simulink model "pwtsimplificado"  (R2025a)
settings: Solver=ode3  StartTime=0.0  StopTime=34  FixedStep=Amostragem/10  RelTol=1e-3
InitFcn:
  | % Suprime os warnings de limite do MFeval. Eles disparam A CADA PASSO quando o pneu
  | % opera fora da faixa do .tir (frenagem forte, baixa velocidade, Fz baixo) e chegam a
  | % custar 10x o tempo de simulacao. Os valores ja sao saturados internamente pelo solver.
  | warning('off','Solver:Limits:Exceeded');
  | warning('off','Solver:CoeffChecks:Ex');
model workspace (MATLAB code in the model file):
  | %% --- Acumulador (lado DC) ----------------------------------------------
  | Bi = 250 ;             % Corrente DC maxima do acumulador (A) - limite de POTENCIA no lado DC.
  |                        %   NAO usar como limite de corrente de fase (ver I_max).
  |                        %   Com 28 kW de pico e EFF ~83%: 234 A @144V -> so 6% de folga.
  | Bv = 168 ;             % Tensao do acumulador (V) - carga cheia (nominal ~144 V)
  | %% --- Motor (identificado a partir das tabelas da folha) ----------------
  | Pnom  = 11000 ;        % Potencia nominal do motor (W)
  | T_max = 94 ;           % Torque maximo/pico 2-min (N*m) - usar na saturacao de Torque_ref
  | Poles = 2 ;            % Numero de PARES de polos (motor de 4 polos -> Poles = 2)
  | Rs  = 0.0165 ;         % Resistencia do estator por fase (Ohm) - folha obs.9: 0.033 de linha /2
  |                        %   (a identificacao usou 0.0144 fixo; diferenca so mexe ~7% no Ki)
  | Rr  = 0.01858 ;        % Resistencia do rotor referida ao estator (Ohm) - IDENTIFICADO
  |                        %   NUNCA usar 0.0248/0.0139: 0.0248 veio do Tau_r=35.5ms
  |                        %   INTERMEDIARIO ERRADO (assumia Kt/Imag antigos); reverter se aparecer.
  | Lls = 7.4763e-5 ;      % Indutancia de dispersao do estator (H) - IDENTIFICADO (Lls=Llr imposto)
  | Llr = 7.4763e-5 ;      % Indutancia de dispersao do rotor (H)   - IDENTIFICADO
  | Lm  = 1.0357e-3 ;      % Indutancia de magnetizacao (H) - IDENTIFICADO (valor LINEAR, fluxo parcial)
  | Ls  = Lls + Lm ;       % Indutancia total do estator (H)  = 1.1105e-3
  | Lr  = Lm + Llr ;       % Indutancia total do rotor (H)    = 1.1105e-3
  | Im  = 0.0071 ;         % Inercia do rotor (kg*m^2). A folha escreve "kgfm2" mas o valor e SI:
  |                        %   carcaca 100 limita o rotor a r<~7cm -> J~0.007-0.01 kg*m^2;
  |                        %   0.0697 (x9.81) exigiria r~12cm, impossivel. [dica: Im=100 trava o rotor]
  | motor_eff = 0.874 ;    % Eficiencia nominal do motor (-) (folha: 87.4% nominal, ~83% no pico)
  | mc_eff    = 0.95 ;     % Eficiencia do inversor (-)
  | %% --- Constantes derivadas do motor -------------------------------------
  | sigma = 1 - (Lm^2)/(Ls*Lr) ;      % Coef. de dispersao total (-)             ~0.1301
  | Tau_r = Lr/Rr ;                   % Constante de tempo do rotor (s)          ~59.8 ms
  |                                   %   Gain "1/Tau_r" embutido no modelo -> 16.73
  | Kt    = (3/2)*Poles*(Lm^2/Lr) ;   % Constante de torque p/ correntes de PICO ~2.898e-3 N*m/A^2
  | Req   = Rs + Rr*((Lm/Lr)^2) ;     % Resistencia equivalente da malha de corrente (Ohm) ~0.0327
  | %% --- Correntes de referencia (PICO de fase) ----------------------------
  | Imag  = 105 ;          % Corrente de magnetizacao (A PICO) - IDENTIFICADA (74 A RMS).
  |                        %   NAO e a "corrente a vazio" da folha (114 RMS = fluxo pleno SATURADO,
  |                        %   fora da regiao linear). Constant "Imag" embutida no modelo -> 105.
  | Idref = Imag ;         % Referencia inicial de corrente do eixo d (A pico)
  | I_max_motor = 242*sqrt(2) ; % Pico 2-min do MOTOR (242 A RMS -> 342.2 pico) - folha
  | I_max_inv   = 257*sqrt(2) ; % Limite AC 1-min do SEVCON Gen5 (257 A RMS -> 363.5 pico)
  | I_max = min(I_max_motor, I_max_inv) ; % limite operativo = o mais restritivo (342.2 pico)
  | % Iq_sat e calculado DINAMICAMENTE no modelo: sqrt(max(I_max^2 - Idref^2, 0))
  | % (limite de corrente vetorial com prioridade ao eixo d - correto)
  | % Torque max alcancavel: Kt*Imag*sqrt(I_max^2-Imag^2) = 99.1 N*m > T_max ✓
  | %% --- Controle discreto / modulacao -------------------------------------
  | Amostragem = 1.25e-4 ; % Periodo de amostragem do controle discreto (s) - 8 kHz
  | Modulation_Target = 0.95 ; % Indice de modulacao alvo (-) - margem antes da sobremodulacao
  | Vmax = (Bv*Modulation_Target)/sqrt(3) ; % Teto de tensao de fase em pico (V)  ~92.1 V
  | % Vq_lim e calculado DINAMICAMENTE no modelo: sqrt(max(Vmax^2 - Vd_sat^2, 0))
  | % (saturacao de tensao vetorial com prioridade ao Vd - correto)
  | c_comp = 1.5 ;         % Compensacao de atraso de angulo (amostras): theta_comp = theta + We*c_comp*Amostragem
  |                        %   SO no caminho de ATUACAO (Inverse Park); a Park direta usa theta puro.
  | %% --- Malha de corrente: ganhos (base p/ parametrizar o SEVCON Gen5) ----
  | wc  = 2*pi*200 ;       % Largura de banda desejada da malha de corrente (rad/s)
  |                        %   regra: wc*Amostragem << 1  (aqui ~0.157, OK)
  | Kp  = sigma*Ls*wc ;    % Ganho proporcional (V/A)        ~0.182
  | Ki  = Req*wc ;         % Ganho integral (V/(A*s))        ~41.0
  | Kaw = Ki/Kp ;          % Anti-windup back-calculation (1/s)  ~226
  |                        %   NUNCA usar 1/(Kp*Amostragem): da Kaw*Ts ~ 2 e diverge.
  |                        %   Conferir: Kaw*Amostragem << 1 (aqui ~0.028)
  | %% --- Field weakening (PI discreto com anti-windup) ---------------------
  | wc_fw     = 2*pi*15 ;              % Banda do laco de FW (rad/s) - MUITO mais lento que wc
  | Fw_margin = 0.95 ;                 % FW age ANTES da saturacao vetorial de tensao.
  |                                    %   NAO criar essa margem baixando Modulation_Target.
  | V_ref_fw  = Vmax*Fw_margin ;       % Referencia do laco de FW (~87.5 V pico de fase)
  | We_base = 2*pi*103 ;               % Ponto de projeto = velocidade base eletrica (rad/s)
  | Kv_fw   = We_base*Ls ;             % Ganho ideal da planta Id->Vmag (~0.719 V/A)
  | Kp_fw  = (1/Kv_fw)/3 ;             % ~0.46 A/V. Margem /3 sobre o ganho ideal.
  |                                    %   HISTORICO: o /10 antigo compensava um BUG ja corrigido:
  |                                    %   a cadeia do Vmag (u^2 -> 1/z -> sqrt -> filtro) rodava na
  |                                    %   taxa do SOLVER (sample time herdado) e lia o PICO do ripple
  |                                    %   intra-amostra (+26 V). Com a cadeia em Amostragem, /3 e
  |                                    %   estavel, sem ciclo limite, e o FW nao fica lento demais.
  | Ki_fw  = Kp_fw*(wc_fw/3) ;         % ~14.6 A/(V*s)
  | Kaw_fw = Ki_fw/Kp_fw ;             % = wc_fw/3 ~ 31.4 1/s
  | Id_min_pu = 0.15 ;                 % Piso de campo (15% de Imag)
  | dImag_max = 0 ;                    % FW so REDUZ campo (saturacao superior = 0)
  | dImag_min = -(1-Id_min_pu)*Imag ;  % Saturacao inferior = -89.25 A (piso garantido AQUI;
  |                                    %   nao por outro Saturation no Id_ref)
  | f_lp_vmag = 50 ;                   % Filtro passa-baixa no V_mag ANTES do somador de erro (Hz)
  | a_vmag    = exp(-2*pi*f_lp_vmag*Amostragem) ; % 0.9615 a 8 kHz
  |                                    %   Discrete TF: [1-a_vmag] / [1 -a_vmag]
  |                                    %   ATENCAO: TODA a cadeia do Vmag (2x Unit Delay, u^2, filtro)
  |                                    %   precisa de Sample Time = Amostragem EXPLICITO nos blocos.
  |                                    %   Herdado (-1) roda na taxa do solver e le o pico do ripple.
  | assert(Kaw_fw*Amostragem < 0.1, 'Kaw_fw alto demais')
  | %% --- Transmissao / roda ------------------------------------------------
  | gear_ratio = 4.45 ;    % Relacao de transmissao (-)
  | trans_eff  = 0.89 ;    % Eficiencia da transmissao (-)
  | Rw = 0.2605 ;          % Raio da roda (m)
  | Iw = 1.20 ;            % Inercia das rodas TRACIONADAS (kg*m^2)
  |                        %   ATENCAO: conferir se ja soma as 2 rodas (Fx do pneu e x2 no Pneu).
  |                        %   Planilha: rodas traseiras = 22 kg o par (11 kg/roda) -> estimativa
  |                        %   ~0.45 kg*m^2/roda (~0.9 o par) + coroa/semieixos. 1.2 e plausivel;
  |                        %   vale medir/calcular no CAD.
  | %% --- Veiculo (dinamica longitudinal) - dados AMP-226 (planilha ago/2026) ---
  | m  = 366 ;             % Massa total com piloto (kg) - aba "Dados Tecnicos"
  |                        %   (a aba "Comportamento do Carro" usa 358.8; diferenca de 2%,
  |                        %    conferir com a equipe qual e a pesagem vigente)
  | g  = 9.81 ;            % Aceleracao da gravidade (m/s^2)
  | air_density = 1.225 ;  % Densidade do ar (kg/m^3)
  | Af = 1.17 ;            % Area frontal (m^2)            - aba "Acoes de aero"
  | Cd = 1.06 ;            % Coef. de arrasto (-)          - aba "Acoes de aero" (CdA = 1.24)
  | Cr = 0.02 ;            % Coef. de resistencia de rolagem (-) - aba "LoadCasesNico" (f = 0.02)
  | %% --- Geometria e cargas (p/ Fz dinamico no pneu) - dados AMP-226 -------
  | L_wb      = 1.56 ;     % Entre-eixos (m)
  | dist_cg_f = 0.804 ;    % Distancia do CG ao eixo DIANTEIRO (m)
  | frac_rear = dist_cg_f/L_wb ; % Fracao de massa no eixo traseiro = 0.5154
  | h_cg      = 0.295 ;    % Altura do CG (m) - calculada; "CG estimado" da planilha = 0.315
  | Fz_rear_static = m*g*frac_rear/2 ; % Carga estatica por roda TRASEIRA = 925.2 N
  |                        %   (Constant "Fz" no subsistema Pneu: era 889 -> usar 925.2,
  |                        %    ou melhor, o Fz dinamico abaixo)
  | ClA_total = 2.11 ;     % Area de lift total (m^2) - tabela de downforce x velocidade da
  |                        %   aba "Acoes de aero" (consistente de 60 a 110 km/h)
  | downforce_rear_share = 0.48 ; % Fracao do downforce no eixo traseiro - ATENCAO: a planilha
  |                        %   tem valores conflitantes (0.45 a 0.58 conforme a aba);
  |                        %   conferir com o subsistema de aero
  | K_transf = (m*h_cg/L_wb)/2 ;       % Ganho ax -> dFz por roda (N por m/s^2) ~34.6
  | K_downf  = 0.5*air_density*ClA_total*downforce_rear_share/2 ; % Ganho Vx^2 -> dFz por roda
  | %% --- Chassi 3-DOF + freios (rev. 5) - ESTIMADOS onde indicado -----------
  | b_cg_r = L_wb - dist_cg_f ;        % Distancia do CG ao eixo TRASEIRO (m) = 0.756
  | Iz  = 120 ;            % Inercia de guinada (kg*m^2) - ESTIMADA (~0.55*m*a*b; tipico FSAE
  |                        %   100-130). Afeta so a rapidez do transitorio de guinada; medir no CAD.
  | Fz_front_static = m*g*(1-frac_rear)/2 ; % Carga estatica por roda DIANTEIRA = 870 N
  | downforce_front_share = 1 - downforce_rear_share ;   % = 0.52
  | K_downf_f = 0.5*air_density*ClA_total*downforce_front_share/2 ; % Vx^2 -> dFz roda dianteira
  | T_brake_max = 1700 ;   % Torque de freio max TOTAL nas rodas (N*m) - ESTIMADO pelo limite de
  |                        %   pneu da planilha (muf=1.8: 1.8*m*g*Rw ~ 1683). Medir o sistema real
  |                        %   (pressao x area de pistao x raio efetivo x mu de pastilha).
  | brake_bias_f = 0.70 ;  % Fracao do freio no eixo dianteiro - ESTIMADA. O ideal a 1.8g seria
  |                        %   ~0.80; conferir a regulagem da balance bar.
  | brake_cut = 0.15 ;     % Pedal de freio acima disso CORTA o torque do motor (brake override,
  | %% --- REGEN (freio regenerativo de lift-off) ----------------------------
  | % Estrategia do carro real: o regen atua sempre que o ACELERADOR esta solto.
  | % O pedal de freio NAO influencia o regen - ele so aciona o freio de atrito,
  | % que soma por cima. Nao ha blending.
  | accel_deadzone = 2 ;   % Pedal de acelerador (%) abaixo disso = "solto" -> regen liga
  | T_regen_max = 94 ;     % Torque max de regen no MOTOR (N*m). O motor/inversor aguentam o
  |                        %   mesmo da tracao; quem limita de verdade e a bateria (Bi_regen).
  | regen_coast = 0.35 ;   % Fracao de T_regen_max com o acelerador totalmente solto (-).
  |                        %   E o ajuste de "sensacao de freio motor". 0.35 -> ~33 N*m.
  | Bi_regen = 60 ;        % <<< CORRENTE MAX DE RECARGA do acumulador (A) - ESTIMADA.
  |                        %   Celulas de Li-ion aceitam bem menos recarga que descarga
  |                        %   (~1-2C contra 5-10C). CONFERIR na folha das celulas e no BMS:
  |                        %   este numero e o que decide quanto regen o carro consegue usar.
  | v_regen_off  = 1.4 ;   % Abaixo desta velocidade o regen e ZERO (m/s ~ 5 km/h).
  |                        %   Exigencia de regra FSAE e tambem fisica: perto da parada o motor
  |                        %   nao gera, e o regen empurraria o carro para tras.
  | v_regen_full = 4.0 ;   % Acima desta velocidade o regen e pleno (m/s). Entre as duas, rampa.
  | w_motor_min  = 20 ;    % Piso de rotacao (rad/s) na divisao do limite de potencia
  | regen_margin = 0.95 ;  % Margem no limite de bateria (-). O limite e de MALHA ABERTA, calculado
  |                        %   pela eficiencia NOMINAL; o ponto real varia. Sem margem, medimos
  |                        %   61 A de pico contra os 60 A de Bi_regen.
  | regen_rate = 200 ;     % Taxa de aplicacao do regen (N*m/s). Sem rampa, tirar o pe da um degrau
  | 
  | %% --- Pose para visualizacao 3D (subsistema "Pose 3D") ------------------
  | % O modelo nao tem dinamica de rolagem nem de arfagem - so 3 GDL no plano.
  | % Para o 3D, roll e pitch sao SINTETIZADOS pelos gradientes quase-estaticos.
  | % Isso e visualizacao, nao dinamica: nao use estes angulos para concluir nada.
  | roll_grad  = 0.7 ;     % Gradiente de rolagem (deg/g) - DA PLANILHA (aba Dados Tecnicos)
  | pitch_grad = 0.5 ;     % Gradiente de arfagem (deg/g) - ESTIMADO. O campo Pitch Gradient
  |                        %   da planilha esta VAZIO; so as anti-geometrias estao preenchidas
  |                        %   (anti-dive 0.312, anti-squat 0.300). Derivar da rigidez ou medir.
  |                        %   de ~113 N*m no torque: solavanco no carro e pico de corrente. O Sevcon
  |                        %   real tambem rampeia. 200 N*m/s -> ~0.17 s para os 33 N*m.
  | %% --- ENTRADA DE DIRECAO (acoes laterais) - subsistema "Direcao" --------
  | % steer_mode escolhe a fonte do angulo de estercamento das rodas dianteiras:
  | %   1 = DEGRAU     : delta_amp entre steer_t0 e steer_t1 (transitorio de guinada)
  | %   2 = SLALOM     : delta_amp*sin(2*pi*steer_freq*(t-steer_t0)) a partir de steer_t0
  | %   3 = RAIO FIXO  : delta = L_wb/R_turn, com rampa de steer_ramp segundos (skidpad)
  | %   4 = WORKSPACE  : usa a timeseries delta_input (dado real, log de pista, MPCC...)
  | steer_mode = 1 ;
  | delta_amp  = 0.03 ;    % Amplitude do estercamento NA RODA (rad). 0.03 rad = 1.72 deg.
  |                        %   Para converter do volante: delta_roda = ang_volante/steer_ratio.
  | steer_t0   = 6.5 ;     % Instante em que a direcao comeca a agir (s)
  | steer_t1   = 9.0 ;     % Fim do degrau, so no modo 1 (s)
  | steer_freq = 0.5 ;     % Frequencia do slalom, so no modo 2 (Hz)
  | R_turn     = 9.125 ;   % Raio da curva, so no modo 3 (m). Skidpad FSAE = 9.125 m.
  | steer_ramp = 1.0 ;     % Tempo de rampa ate o esterco pleno no modo 3 (s)
  | delta_max  = 0.35 ;    % Limite mecanico do estercamento na roda (rad) ~20 deg
  | steer_rate_max = 3.0 ; % Velocidade maxima de esterco na roda (rad/s) - limita o degrau,
  |                        %   representa piloto + sistema de direcao (nao ha degrau perfeito).
  | delta_input = timeseries([0;0],[0;1000]) ;  % Modo 4: substitua por sua timeseries.
  |                        %   Ex: delta_input = timeseries(ang_rad, tempo_s);
  |                        %   como a VCU real). Gate = sat(1 - pedal/brake_cut, 0, 1).
  | %% --- Pneu dianteiro analitico (Magic Formula calibrada no Avon 9760) ----
  | % Coeficientes extraidos do PROPRIO .tir rodando mfeval offline (fit com erro <0.5%).
  | % Por que analitico e nao um 2o bloco MFeval: o MFeval em modo "non-linear transients"
  | % com roda livre em baixa velocidade itera internamente e deixou a simulacao 52x mais
  | % lenta (0.12 vs 6.3 sim-s/min). O eixo dianteiro nao recebe torque de tracao, entao
  | % a Magic Formula com elipse de atrito e suficiente e roda compilada.
  | Ca_c1 = 36392 ;        % C_alpha(Fz) = Ca_c1*sin(2*atan(Fz/Ca_c2))  [N/rad, por roda]
  | Ca_c2 = 1474 ;
  | mu_a  = 2.6537 ;       % mu_y(Fz) = mu_a + mu_b*Fz  (sensibilidade de carga)
  | mu_b  = -2.225e-4 ;
  | Cf_shape = 1.3 ;       % Fator de forma C da Magic Formula (tipico de pneu de competicao)
  | Vx_min_tire = 1.0 ;    % Piso de Vx nas divisoes do modelo de pneu (m/s)
  | mu_scale = 1.0 ;       % <<< DERATING DE PISTA - vale para os DOIS eixos.
  |                        %   O .tir da mu ~2.45 (dado de bancada, estilo TTC). A planilha do
  |                        %   carro usa mu 1.7-1.8 (pista real) -> mu_scale ~0.70.
  |                        %   Entra no eixo dianteiro E no muRoad do MFeval traseiro.
  | Iw_f = 0.9 ;           % Inercia do PAR de rodas dianteiras (kg*m^2) - ESTIMADA. NAO usada
  |                        %   no modelo analitico (sem estado de roda); fica p/ referencia.
  | % Fz dinamico por roda traseira - JA FIADO no subsistema Pneu:
  | %   Fz_rear = Fz_rear_static + K_transf*ax_filtrado + K_downf*Vx^2
  | %   ax vem do Goto global "ax" (saida do ganho 1/m no subsistema Veiculo),
  | %   filtrado por 1/(0.1s+1) - quebra o laco algebrico Fz->Fx->ax->Fz e representa
  | %   a dinamica da suspensao na transferencia de carga.
  | %% --- Condicoes iniciais dos sinais -------------------------------------
  | % Evitam divisao por zero no controlador e singularidade de escorregamento
  | % do modelo de pneu (MFeval) em Vx = 0.
  | Velocity    = 0.1 ;    % Velocidade inicial do veiculo (m/s)
  | Wheel_Speed = 1 ;      % Velocidade angular inicial da roda (rad/s)
  | Iqref = 0.1 ;          % Valor inicial da referencia de corrente do eixo q (A)
  | Vd    = 0.1 ;          % Valor inicial da tensao do eixo d (V)
  | Vq    = 0.1 ;          % Valor inicial da tensao do eixo q (V)
  | %% --- Pneu (MFeval) -----------------------------------------------------
  | % Arquivo .tir procurado a partir da pasta do modelo (data/ ou ao lado do .slx),
  | % depois no path do MATLAB - nada de caminho absoluto, roda em qualquer maquina.
  | tirNome = 'Avon_9760_Round_2.tir';
  | try, raizModelo = fileparts(get_param('pwtsimplificado','FileName')); catch, raizModelo = pwd; end
  | tirFile = '';
  | for c = {fullfile(raizModelo,'data',tirNome), fullfile(raizModelo,tirNome), which(tirNome)}
  |     if ~isempty(c{1}) && isfile(c{1}), tirFile = c{1}; break, end
  | end
  | assert(~isempty(tirFile), 'Arquivo %s nao encontrado em %s/data nem no path do MATLAB.', tirNome, raizModelo);
  | tirParams = mfeval.readTIR(tirFile);
  | %% --- Verificacoes rapidas (rodar sempre que mudar parametros) ----------
  | fprintf('--- Verificacoes ---\n');
  | fprintf('Kaw*Ts   = %.4f | wc*Ts = %.4f  (ambos << 1)\n', Kaw*Amostragem, wc*Amostragem);
  | fprintf('sigma    = %.4f (esperado 0.130) | Tau_r = %.1f ms (esperado 59.8 - se der ~35, Rr esta ERRADO)\n', sigma, Tau_r*1e3);
  | fprintf('Kt = %.4g (esperado 2.898e-3) | Req = %.4g\n', Kt, Req);
  | fprintf('Kp = %.3f V/A | Ki = %.1f V/(A*s) | Kaw = %.1f 1/s\n', Kp, Ki, Kaw);
  | fprintf('FW: Kp_fw = %.3f | Ki_fw = %.2f | Kaw_fw = %.2f | dImag_min = %.2f\n', Kp_fw, Ki_fw, Kaw_fw, dImag_min);
  | fprintf('Vmax = %.1f V | V_ref_fw = %.1f V | Imag = %.0f A pico | I_max = %.1f A pico\n', Vmax, V_ref_fw, Imag, I_max);
  | fprintf('Torque max alcancavel = %.1f N*m (deve ser > T_max = %.0f)\n', Kt*Imag*sqrt(I_max^2-Imag^2), T_max);
  | fprintf('--- Alvos de aceitacao (tabelas da folha, NAO o cabecalho) ---\n');
  | Iq35 = 35/(Kt*Imag); Iq94 = 94/(Kt*Imag);
  | fprintf('35 N*m: I = %.1f A RMS (folha sub-base: 110-111) | slip = %.2f Hz (folha: 3.0-3.3)\n', ...
  |         sqrt(Imag^2+Iq35^2)/sqrt(2), Iq35/(Tau_r*Imag)/(2*pi));
  | fprintf('94 N*m: I = %.1f A RMS (folha: 240; ~4%% de folga = saturacao/ferro) | slip = %.2f Hz (folha: ~8)\n', ...
  |         sqrt(Imag^2+Iq94^2)/sqrt(2), Iq94/(Tau_r*Imag)/(2*pi));
  | fprintf('Joelho de FW esperado: ~2970 RPM a torque pleno | Id_ref >= %.0f A ate 4800 RPM\n', 0.55*Imag);
  | fprintf('P_DC: disponivel %.1f kW | pico estimado %.1f kW (com EFF pico 0.83)\n', Bv*Bi/1e3, 28/0.83);
  | fprintf('--- Chassi 3-DOF / freios ---\n');
  | fprintf('Iz = %g kg*m^2 (estimado) | Fz est.: diant %.0f N / tras %.0f N\n', Iz, Fz_front_static, Fz_rear_static);
  | fprintf('Freio: %.0f N*m total, bias %.0f%% diant -> Fx max %.0f N = %.2f g\n', ...
  |         T_brake_max, 100*brake_bias_f, T_brake_max/Rw, T_brake_max/Rw/(m*g));
  | fprintf('Pneu: mu(Fz est. tras) = %.2f | C_alpha = %.0f N/rad | mu_scale = %.2f\n', ...
  |         mu_scale*(mu_a + mu_b*Fz_rear_static), Ca_c1*sin(2*atan(Fz_rear_static/Ca_c2)), mu_scale);
  | K_us_est = (m*g*(1-frac_rear))/(2*Ca_c1*sin(2*atan(Fz_front_static/Ca_c2))) ...
  |          - (m*g*frac_rear)/(2*Ca_c1*sin(2*atan(Fz_rear_static/Ca_c2)));
  | if K_us_est > 0, comport = 'subesterco'; else, comport = 'sobreesterco'; end
  | fprintf('Gradiente de esterco (estatico) = %+.5f rad/(m/s^2) -> %s leve\n', K_us_est, comport);
  | %% =======================================================================
  | %  NOTA - Arquitetura de pneu: por que MFeval so no TRASEIRO, em steady state
  | %  -----------------------------------------------------------------------
  | %  Medicoes feitas neste modelo (12 s, fixed-step ode3, passo Amostragem/10):
  | %
  | %    configuracao                                      regime normal | frenagem
  | %    2x MFeval (nao-linear transients)                     0.12      |   --
  | %    MFeval tras (nao-linear) + analitico diant            2.8       |  0.21
  | %    MFeval tras (STEADY STATE) + analitico + warn off     5.4       |  2.4
  | %                                                       [sim-s por minuto]
  | %
  | %  1) NUNCA use dois blocos MFeval. O custo nao e 2x, e ~50x: a roda dianteira
  | %     livre em baixa velocidade cai fora da faixa do .tir e o solver entra no
  | %     caminho caro (sem laco algebrico e sem colapso de passo - e custo bruto).
  | %
  | %  2) A CAUSA RAIZ do travamento em baixa velocidade sao os LIMIT CHECKS.
  | %     mfeval.Solver/fullCPI fixa useMode = 111 (limit checks SEMPRE ligados) e
  | %     nao ha opcao no mask para desligar. Quando um limite e excedido (Vx<VXLOW=1,
  | %     Fz<FZMIN=222, |kappa|>KPUMAX=0.52), o solver chama warning() A CADA PASSO.
  | %     Medido: o warning custa 2x e o caminho fora-de-limite mais 2-4x.
  | %     Solucao (no InitFcn do modelo, ja configurado):
  | %         warning('off','Solver:Limits:Exceeded');
  | %         warning('off','Solver:CoeffChecks:Ex');
  | %     Efeito medido na frenagem: 0.21 -> 2.4 sim-s/min (11x). Nao altera
  | %     resultado nenhum: os valores ja sao saturados internamente pelo solver.
  | %
  | %  3) Dynamics = "1 steady state" no lugar de "3 non-linear transients":
  | %     2x mais rapido e resultado IDENTICO neste modelo
  | %     (psi_dot 0.5085 vs 0.5090 | Te 93.87 vs 93.9 | frenagem -1.09 g nos dois).
  | %     A doc do MFeval recomenda passo <=0.00025 s para transientes nao-lineares
  | %     e <=0.01 s para steady state; o nosso passo (1.25e-5) atende com folga aos
  | %     dois. Volte para nao-linear transients SO se for estudar transitorio rapido
  | %     de pneu (controle de tracao, ABS de alta banda) - ai o custo se justifica.
  | %
  | %  4) Por que manter MFeval no traseiro: e o eixo que transmite TODO o torque do
  | %     motor, entao o Fx(kappa) de escorregamento combinado do Pacejka e justamente
  | %     o que define largada, patinacao e quanto dos 94 N*m chega ao chao. E a
  | %     referencia validada com os dados reais do Avon. O dianteiro nao recebe
  | %     tracao, entao a MF analitica calibrada no mesmo .tir basta (validada:
  | %     psi_dot dentro de 2.6% do modelo bicicleta teorico).
  | 
  | %% ==== PILOTO DE PISTA (rev. 11) ====
  | %  Acrescentado por add_piloto.m. Tudo aqui e OPCIONAL:
  | %     steer_mode = 5  ->  estercamento por pure pursuit
  | %     piloto_on  = 1  ->  acelerador pelo alvo de velocidade
  | %  Com os dois em zero o modelo se comporta exatamente como antes.
  | pistaArq = fullfile(raizModelo,'data','pista_amp226.mat');   % raizModelo vem do bloco do pneu
  | if ~isfile(pistaArq), pistaArq = which('pista_amp226.mat'); end
  | if ~isempty(pistaArq) && isfile(pistaArq)
  |     pista_ = load(pistaArq);
  |     pista_ = pista_.pista;
  |     trk_passo = 0.5;
  |     s_    = transpose(0 : trk_passo : pista_.Lap - trk_passo);
  |     trk_x = interp1(pista_.s, pista_.x,     s_);
  |     trk_y = interp1(pista_.s, pista_.y,     s_);
  |     trk_k = interp1(pista_.s, pista_.kappa, s_);
  |     clear pista_ s_
  | else
  |     % Sem pista no disco o piloto nao tem para onde ir. Tabelas minimas so
  |     % para o modelo continuar compilando com steer_mode ~= 5.
  |     trk_passo = 0.5;  trk_x = [0;1];  trk_y = [0;0];  trk_k = [0;0];
  | end
  | 
  | pp_Ld_min  = 4.0;    % mira minima [m] - abaixo disso o carro serpenteia
  | pp_Ld_k    = 0.55;   % a mira cresce com a velocidade: Ld = pp_Ld_k*Vx
  | pp_v_max   = 22.0;   % teto de velocidade [m/s]
  | pp_ay_max  = 9.0;    % aceleracao lateral admitida [m/s^2] ~ 0,9 g
  | pp_kp_v    = 0.35;   % ganho do acelerador por erro de velocidade
  | pp_kp_b    = 0.30;   % ganho do FREIO por excesso de velocidade [1/(m/s)]
  | pp_v_banda = 0.8;    % banda morta antes de pisar no freio [m/s]. Abaixo dela
  |                      % quem desacelera e o regen de lift-off, sem atrito.
  | pp_frn_max = 0.90;   % pedal de freio maximo. E FRACAO 0..1, escala diferente
  |                      % do acelerador - o Brake_pedal do modelo ja e normalizado.
  | pp_prev    = 12.0;   % quantos metros a frente olhar a curvatura
  | pp_Ts      = 0.01;   % taxa do piloto [s] - 100 Hz
  | pp_ped_max = 100;    % fundo de escala do acelerador. NAO e 0..1: o "pedal"
  |                      % deste modelo e requisicao de TORQUE (lookup [0:94]).
  | piloto_on  = 1;      % 0 = quem manda no acelerador e o Signal Builder
  | steer_mode = 5;      % 5 = pure pursuit
  | %% ==== fim do piloto ====
undefined symbols (not defined in the file): DiscIntNeverNeededParam, dspblkCoreblockFVToolHelper, gcbh, sigbuilder_block, Vq_lim
libraries: mcbeeMathTransformLib x4, spsControlledVoltageSourceLib x3, spsGroundLib x3, simulink x2, spsAsynchronousMachineSIUnitsLib x1, spspowerguiLib x1, mfeval_LIB x1
(part 1 of 2)
settings Model: Creator=gabox  LastModifiedBy=gabox
settings ModelReferenceCC: EnableRefExpFcnMdlSchedulingChecks=on
settings RTWCC: GPUComputeCapability=3.5

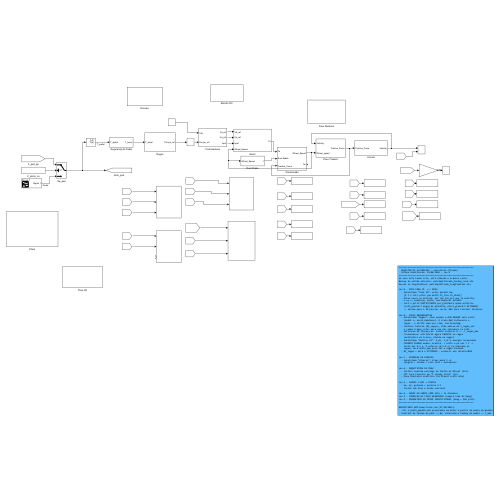
[thumbnail: Simulink's stored preview of the top-level diagram]
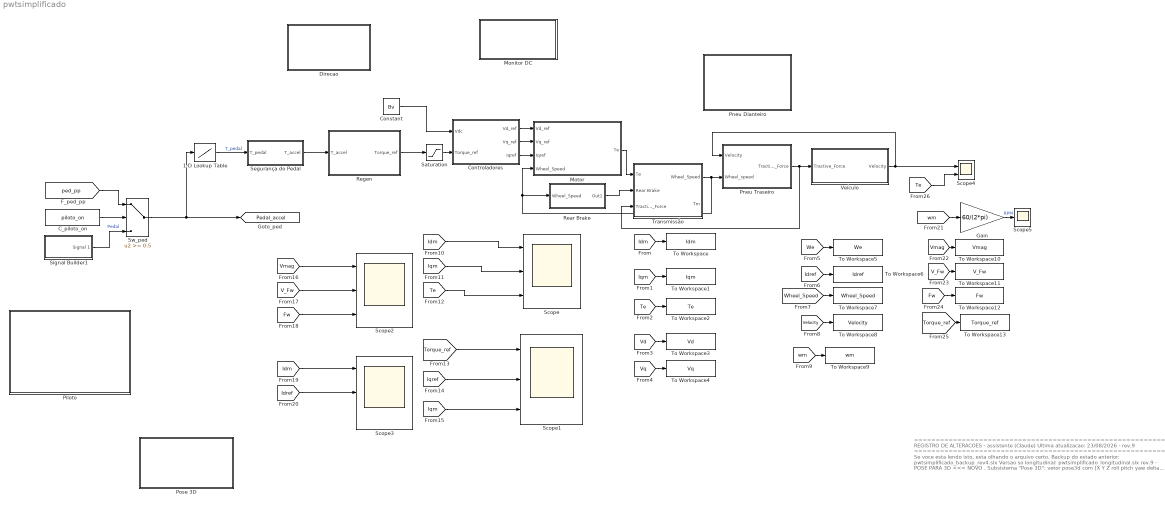
== system pwtsimplificado ==
  note: ==========================================================
      |   REGISTRO DE ALTERACOES - assistente (Claude)
      |   Ultima atualizacao: 23/08/2026 - rev.9
      | ==========================================================
      | Se voce esta lendo isto, esta olhando o arquivo certo.
      | Backup do estado anterior: pwtsimplificado_backup_rev4.slx
      | Versao so longitudinal: pwtsimplificado_longitudinal.slx
      |
      | rev.9 - POSE PARA 3D  <<< NOVO
      |   . Subsistema "Pose 3D": vetor pose3d com
      |     [X Y Z roll pitch yaw delta th_tras th_diant]
      |   . Gotos novos no Veiculo: psi (do Int_psi que ja existia)
      |     e ay (= somaFy/m, exato, sem duplicar estado)
      |   . roll e pitch SINTETIZADOS por gradiente quase-estatico
      |     (roll_grad=0.7 deg/g da planilha; pitch_grad=0.5 ESTIMADO)
      |     -> servem para o 3D parecer certo, NAO para concluir dinamica
      |
      | rev.8 - FREIO REGENERATIVO
      |   . Subsistema "Regen": atua quando o ACELERADOR esta solto
      |     (pedal <= accel_deadzone). O freio NAO influencia o
      |     regen - o atrito soma por cima, sem blending.
      |   . Limites: bateria (Bi_regen), fade abaixo de v_regen_off
      |     e rampa (regen_rate) para nao dar solavanco no lift.
      |   . Saturacao do Torque_ref: limite inferior 0 -> -T_regen_max
      |   . Transmissao: eficiencia agora INVERTE no regen
      |     (multiplica em tracao, divide em regen)
      |   . Subsistema "Monitor DC": P_dc, I_dc e energia recuperada
      |   . CENARIO PADRAO mudou: acelera -> solta o pe aos 7 s ->
      |     freia aos 9,5 s. O esterco (6,5-9 s) se sobrepoe ao
      |     regen; zere delta_amp para ler o regen isolado.
      |   . Bi_regen = 60 A e ESTIMADO - conferir nas celulas/BMS
      |
      | rev.7 - ENTRADAS DE DIRECAO
      |   . Subsistema "Direcao": steer_mode 1..4
      |     (degrau / slalom / raio fixo / workspace)
      |
      | rev.6 - ARQUITETURA DE PNEU
      |   . InitFcn suprime warnings de limite do MFeval (11x)
      |   . CPI tyre traseiro em "1 steady state" (2x)
      |   . Pneu dianteiro analitico (2o MFeval custa ~50x)
      |
      | rev.5 - CHASSI 3-DOF + FREIOS
      |   . Vx, Vy, guinada + posicao X-Y
      |   . Freios com bias e brake override
      |
      | rev.4 - DADOS DO CARRO (AMP-226) + Fz dinamico
      | rev.3 - CORRECAO DO FIELD WEAKENING (sample time do Vmag)
      | rev.2 - PARAMETROS DO MOTOR IDENTIFICADOS (Imag = 105 pico)
      | ==========================================================
      |
      | REPOSITORIO AMP-Powertrain-sim (27/10/2026):
      | . .tir e pista_amp226.mat procurados em data/ a partir da pasta do modelo
      | . Constant da tensao do pack -> Bv; saturacao e lookup do pedal -> T_max
  1-D Lookup Table : Lookup_n-D  NumberOfTableDimensions=1  BreakpointsForDimension1=[0 T_max]  Table=[0 T_max]  InternalRulePriority=Speed  RndMeth=Simplest
  C_piloto_on : Constant  Value=piloto_on
  Constant : Constant  Value=Bv
  Controladores : Subsystem
  Direcao : Subsystem
  Gain : Gain  Gain=60/(2*pi)
  Monitor DC : Subsystem
  Motor : Subsystem
  Piloto : Subsystem
  Pneu Dianteiro : Subsystem
  Pneu Traseiro : Subsystem
  Pose 3D : Subsystem
  Rear Brake : Subsystem
  Regen : Subsystem
  Saturation : Saturate  UpperLimit=T_max  LowerLimit=-T_regen_max
  Scope{,1..3} (4 alike) : Scope  NumInputPorts=3
      Scope settings: ActiveDisplayYMinimum=-41.513941391291461  ActiveDisplayYMaximum=373.62547252162324  DataLoggingVariableName=ScopeData2
      Scope1 settings: ActiveDisplayYMinimum=-1  ActiveDisplayYMaximum=1  DataLoggingVariableName=ScopeData3
      Scope2 settings: ActiveDisplayYMinimum=-173.12729270620673  ActiveDisplayYMaximum=187.77269241633141  DataLoggingVariableName=ScopeData4
      Scope3 settings: ActiveDisplayYMinimum=-22.382704849224424  ActiveDisplayYMaximum=201.44434364301986
  Scope4 : Scope  NumInputPorts=2
      settings: ActiveDisplayYMinimum=-13.525918315638208  ActiveDisplayYMaximum=121.7332648407439  DataLoggingVariableName=ScopeData5
  Scope5 : Scope
      settings: DataLoggingVariableName=ScopeData6
  Segurança do Pedal : Subsystem
  Signal Builder1 : Subsystem  Tag=STV Subsys  LoadFcn=sigbuilder_block('load');  StartFcn=sigbuilder_block('start');  StopFcn=sigbuilder_block('stop');  ClipboardFcn=sigbuilder_block('clipboard');  mask(Sigbuilder block){tuvar=[0:10]}
      mask help: Simulink:masks:SigbuilderBlock_MD
      mask init:
      | if ~strcmp(get_param(bdroot(gcbh),'SimulationStatus'),'stopped') tuvar = sigbuilder_block('maskInit'); end
      settings: CopyFcn=sigbuilder_block('copy');  DeleteFcn=sigbuilder_block('delete');  ModelCloseFcn=sigbuilder_block('modelClose');  PreSaveFcn=sigbuilder_block('preSave');  PauseFcn=sigbuilder_block('pause');  ContinueFcn=sigbuilder_block('continue');  NameChangeFcn=sigbuilder_block('namechange');  OpenFcn=sigbuilder_block('open',[252.75 107.25 644.25 387.75 ]);  CloseFcn=sigbuilder_block('close');
      mask Display: plot(0, 0, 100, 100,[2, 2, 32, 32, 2], [68, 8, 8, 68, 68],[32, 2], [38, 38], [32, 19, 2],[53, 60, 44], [32, 17, 17, 2],[16, 16, 31, 31]);txt = getActiveGroup(gcbh);text(2, 100, txt,'verticalAlignment', 'top');
  Sw_ped : Switch  Threshold=0.5
  To Workspace : ToWorkspace  VariableName=Idm  SaveFormat=Timeseries  SampleTime=Amostragem
  To Workspace1 : ToWorkspace  VariableName=Iqm  SaveFormat=Timeseries  SampleTime=Amostragem
  To Workspace10 : ToWorkspace  VariableName=Vmag  SaveFormat=Timeseries  SampleTime=Amostragem
  To Workspace11 : ToWorkspace  VariableName=V_Fw  SaveFormat=Timeseries  SampleTime=Amostragem
  To Workspace12 : ToWorkspace  VariableName=Fw  SaveFormat=Timeseries  SampleTime=Amostragem
  To Workspace13 : ToWorkspace  VariableName=Torque_ref  SaveFormat=Timeseries  SampleTime=Amostragem
  To Workspace2 : ToWorkspace  VariableName=Te  SaveFormat=Timeseries  SampleTime=Amostragem
  To Workspace3 : ToWorkspace  VariableName=Vd  SaveFormat=Timeseries  SampleTime=Amostragem
  To Workspace4 : ToWorkspace  VariableName=Vq  SaveFormat=Timeseries  SampleTime=Amostragem
  To Workspace5 : ToWorkspace  VariableName=We  SaveFormat=Timeseries  SampleTime=Amostragem
  To Workspace6 : ToWorkspace  VariableName=Idref  SaveFormat=Timeseries  SampleTime=Amostragem
  To Workspace7 : ToWorkspace  VariableName=Wheel_Speed  SaveFormat=Timeseries  SampleTime=Amostragem
  To Workspace8 : ToWorkspace  VariableName=Velocity  SaveFormat=Timeseries  SampleTime=Amostragem
  To Workspace9 : ToWorkspace  VariableName=wm  SaveFormat=Timeseries  SampleTime=Amostragem
  Transmissão : Subsystem
  Veículo : Subsystem
  tag scope: Pedal_accel=global
  wires:
  Transmissão/1(Wheel_Speed) -> Pneu Traseiro/2(Wheel_speed), Motor/4(Wheel_Speed), Rear Brake/1(Wheel_Speed)
  Veículo/1(Velocity) -> Pneu Traseiro/1(Velocity), Scope4/1
  Motor/1(Te) -> Transmissão/1(Te)
  Pneu Traseiro/1(Tractive_Force) -> Veículo/1(Tractive_Force), Transmissão/3(Tractive_Force)
  Controladores/1(Vd_ref) -> Motor/1(Vd_ref)
  Controladores/2(Vq_ref) -> Motor/2(Vq_ref)
  Constant/1 -> Controladores/1(Vdc)
  Saturation/1 -> Controladores/2(Torque_ref)
  Controladores/3(Iqref) -> Motor/3(Iqref)
  [Idm] -> To Workspace/1
  [Iqm] -> To Workspace1/1
  [Vd] -> To Workspace3/1
  [Te] -> To Workspace2/1
  [Vq] -> To Workspace4/1
  [Idref] -> To Workspace6/1
  [We] -> To Workspace5/1
  [Wheel_Speed] -> To Workspace7/1
  [Velocity] -> To Workspace8/1
  [wm] -> To Workspace9/1
  [Idm] -> Scope/1
  [Iqm] -> Scope/2
  [Te] -> Scope/3
  [Torque_ref] -> Scope1/1
  [Iqref] -> Scope1/2
  [Iqm] -> Scope1/3
  [Fw] -> Scope2/3
  [Vmag] -> Scope2/1
  [V_Fw] -> Scope2/2
  [Idm] -> Scope3/1
  [Idref] -> Scope3/2
  [Vmag] -> To Workspace10/1
  [V_Fw] -> To Workspace11/1
  [Fw] -> To Workspace12/1
  [Torque_ref] -> To Workspace13/1
  1-D Lookup Table/1 -> Segurança do Pedal/1(T_pedal)  "T_pedal"
  Rear Brake/1(Out1) -> Transmissão/2(Rear Brake)
  [Te] -> Scope4/2
  Gain/1 -> Scope5/1  "RPM"
  [wm] -> Gain/1
  Segurança do Pedal/1(T_accel) -> Regen/1(T_accel)
  Regen/1(Torque_ref) -> Saturation/1
  [ped_pp] -> Sw_ped/1
  C_piloto_on/1 -> Sw_ped/2
  Signal Builder1/1(Signal 1) -> Sw_ped/3  "Pedal"
  Sw_ped/1 -> 1-D Lookup Table/1, [Pedal_accel]

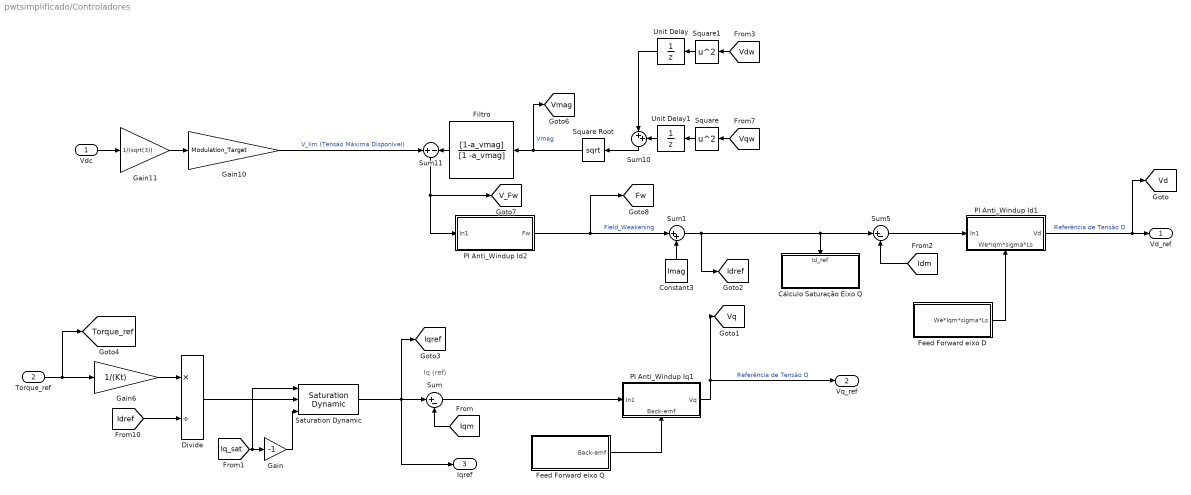
== system pwtsimplificado/Controladores ==
  note: Iq (ref)
  Vdc : Inport
  Torque_ref : Inport  Port=2
  Constant3 : Constant  Value=Imag
  Cálculo Saturação Eixo Q : Subsystem
      settings: PortSchema="{\"entries\":[{\"content\":{\"sides\":[{\"content\":{},\"type\":\"ConnectorPlacement.EquallySpacedRectSide\",\"uuid\":\"7f7fb8a8-2f6b-4961-9c00-1f4e2fc5b775\"},{\"content\":{\"side\":\"RIGHT\"},\"type\":\"ConnectorPlacement.EquallySpacedRectSide\",\"uuid\":\"99257d35-6f07-42ed-a793-bbf32f624519\"},{\"content\":{\"connectorIds\":[\"In1\"],\"side\":\"TOP\"},\"type\":\"ConnectorPlacement.EquallySpacedRectSide\",\"uuid\":\"78fef148-479c-4404-810b-4f212cfc0a7c\"}]},\"type\":\"ConnectorPlacement.EquallySpacedConnector\",\"uuid\":\"0774de6e-bcfc-41a2-9f60-6d7989875326\"}],\"packageUris\":[\"http://schema.mathworks.com/mf0/Connector/R2020b\"],\"version\":\"1.0\"}"
  Divide : Product  Inputs=*/
  Feed Forward eixo D : Subsystem
  Feed Forward eixo Q : Subsystem
  Filtro : DiscreteTransferFcn  LoadFcn=dspblkCoreblockFVToolHelper(gcbh,'load');  Numerator=[1-a_vmag]  Denominator=[1 -a_vmag]  SampleTime=Amostragem
      settings: CopyFcn=dspblkCoreblockFVToolHelper(gcbh,'copy');  DeleteFcn=dspblkCoreblockFVToolHelper(gcbh,'close');  ModelCloseFcn=dspblkCoreblockFVToolHelper(gcbh,'close');  PreSaveFcn=dspblkCoreblockFVToolHelper(gcbh,'presave');  PostSaveFcn=dspblkCoreblockFVToolHelper(gcbh,'postsave');  CloseFcn=dspblkCoreblockFVToolHelper(gcbh,'close');
  Gain : Gain  Gain=-1
  Gain10 : Gain  Gain=Modulation_Target
  Gain11 : Gain  Gain=1/(sqrt(3))
  Gain6 : Gain  Gain=1/(Kt)
  PI Anti_Windup Id1 : Subsystem
      settings: PortSchema="{\"entries\":[{\"content\":{\"sides\":[{\"content\":{\"connectorIds\":[\"In1\"]},\"type\":\"ConnectorPlacement.EquallySpacedRectSide\",\"uuid\":\"0de77585-2e0a-4dcb-a42d-23ce97468db2\"},{\"content\":{\"connectorIds\":[\"Out1\"],\"side\":\"RIGHT\"},\"type\":\"ConnectorPlacement.EquallySpacedRectSide\",\"uuid\":\"33b7113f-9ed7-41a2-ab15-fe3179c74bc1\"},{\"content\":{\"connectorIds\":[],\"side\":\"TOP\"},\"type\":\"ConnectorPlacement.EquallySpacedRectSide\",\"uuid\":\"80085514-688f-4280-b0ee-d4b30b84859c\"},{\"content\":{\"connectorIds\":[\"In2\"],\"side\":\"BOTTOM\"},\"type\":\"ConnectorPlacement.EquallySpacedRectSide\",\"uuid\":\"df22b881-1b5e-45ae-891f-eebf20510deb\"}]},\"type\":\"ConnectorPlacement.EquallySpacedConnector\",\"uuid\":\"87582b80-d1ad-469a-97fa-00e7f61ced2e\"}],\"packageUris\":[\"http://schema.mathworks.com/mf0/Connector/R2020b\"],\"version\":\"1.0\"}"
  PI Anti_Windup Id2 : Subsystem
  PI Anti_Windup Iq1 : Subsystem
      settings: PortSchema="{\"entries\":[{\"content\":{\"sides\":[{\"content\":{\"connectorIds\":[\"In1\"]},\"type\":\"ConnectorPlacement.EquallySpacedRectSide\",\"uuid\":\"0de77585-2e0a-4dcb-a42d-23ce97468db2\"},{\"content\":{\"connectorIds\":[\"Out1\"],\"side\":\"RIGHT\"},\"type\":\"ConnectorPlacement.EquallySpacedRectSide\",\"uuid\":\"33b7113f-9ed7-41a2-ab15-fe3179c74bc1\"},{\"content\":{\"connectorIds\":[],\"side\":\"TOP\"},\"type\":\"ConnectorPlacement.EquallySpacedRectSide\",\"uuid\":\"80085514-688f-4280-b0ee-d4b30b84859c\"},{\"content\":{\"connectorIds\":[\"In2\"],\"side\":\"BOTTOM\"},\"type\":\"ConnectorPlacement.EquallySpacedRectSide\",\"uuid\":\"df22b881-1b5e-45ae-891f-eebf20510deb\"}]},\"type\":\"ConnectorPlacement.EquallySpacedConnector\",\"uuid\":\"87582b80-d1ad-469a-97fa-00e7f61ced2e\"}],\"packageUris\":[\"http://schema.mathworks.com/mf0/Connector/R2020b\"],\"version\":\"1.0\"}"
  Saturation Dynamic : simulink/Discontinuities/Saturation Dynamic  OutMin=[]  OutMax=[]  OutDataTypeStr=Inherit: Same as second input  OutDataType=fixdt(1, 16)  OutScaling=2^-10  DoSatur=off
  Square : Math  Operator=square
  Square Root : Sqrt
  Square1 : Math  Operator=square
  Sum : Sum  Inputs=|+-
  Sum1 : Sum  Inputs=|++
  Sum10 : Sum  Inputs=|++
  Sum11 : Sum  Inputs=+|-
  Sum5 : Sum  Inputs=|+-
  Unit Delay : UnitDelay  SampleTime=Amostragem  HasFrameUpgradeWarning=on
  Unit Delay1 : UnitDelay  SampleTime=Amostragem  HasFrameUpgradeWarning=on
  Vd_ref : Outport
  Vq_ref : Outport  Port=2
  Iqref : Outport  Port=3
  tag scope: Fw=global, Idref=global, Iqref=global, Torque_ref=global, V_Fw=global, Vd=global, Vmag=global, Vq=global
  wires:
  PI Anti_Windup Id2/1(Fw) -> [Fw], Sum1/1  "Field_Weakening"
  Vdc/1 -> Gain11/1
  Sum5/1 -> PI Anti_Windup Id1/1(In1)
  Sum11/1 -> [V_Fw], PI Anti_Windup Id2/1(In1)
  Gain11/1 -> Gain10/1
  Sum/1 -> PI Anti_Windup Iq1/1(In1)
  PI Anti_Windup Iq1/1(Vq) -> Vq_ref/1, [Vq]  "Referência de Tensão Q"
  Gain10/1 -> Sum11/1  "V_lim (Tensão Máxima Disponível)"
  [Idm] -> Sum5/2
  PI Anti_Windup Id1/1(Vd) -> [Vd], Vd_ref/1  "Referência de Tensão D"
  Square Root/1 -> Filtro/1, [Vmag]  "Vmag"
  Constant3/1 -> Sum1/2
  Sum1/1 -> Sum5/1, Cálculo Saturação Eixo Q/1(Id_ref), [Idref]
  Sum10/1 -> Square Root/1
  Unit Delay1/1 -> Sum10/2
  Unit Delay/1 -> Sum10/1
  Square/1 -> Unit Delay1/1
  Square1/1 -> Unit Delay/1
  [Iqm] -> Sum/2
  Torque_ref/1 -> [Torque_ref], Gain6/1
  [Idref] -> Divide/2
  Gain6/1 -> Divide/1
  Feed Forward eixo D/1(We*Iqm*sigma*Ls) -> PI Anti_Windup Id1/2(We*Iqm*sigma*Ls)
  Feed Forward eixo Q/1(Back-emf) -> PI Anti_Windup Iq1/2(Back-emf)
  Divide/1 -> Saturation Dynamic/2
  Saturation Dynamic/1 -> [Iqref], Iqref/1, Sum/1
  [Iq_sat] -> Saturation Dynamic/1, Gain/1
  Gain/1 -> Saturation Dynamic/3
  [Vdw] -> Square1/1
  [Vqw] -> Square/1
  Filtro/1 -> Sum11/2

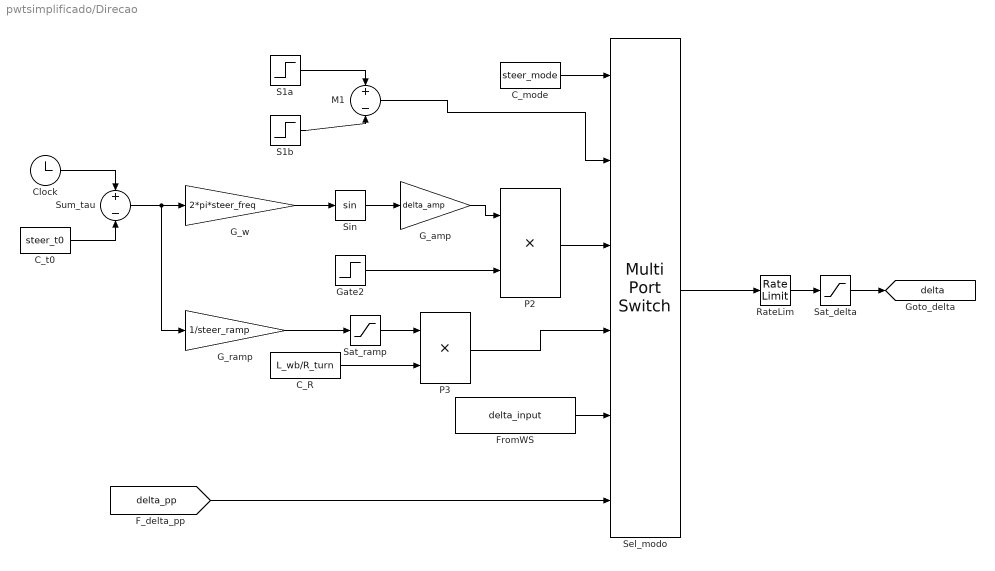
== system pwtsimplificado/Direcao ==
  C_R : Constant  Value=L_wb/R_turn
  C_mode : Constant  Value=steer_mode
  C_t0 : Constant  Value=steer_t0
  Clock : Clock
  FromWS : FromWorkspace  VariableName=delta_input  OutputAfterFinalValue=Holding final value
  G_amp : Gain  Gain=delta_amp
  G_ramp : Gain  Gain=1/steer_ramp
  G_w : Gain  Gain=2*pi*steer_freq
  Gate2 : Step  Time=steer_t0  SampleTime=0
  M1 : Sum  Inputs=+-
  P2 : Product
  P3 : Product
  RateLim : RateLimiter  RisingSlewLimit=steer_rate_max  FallingSlewLimit=-steer_rate_max  SampleTimeMode=inherited
  S1a : Step  Time=steer_t0  After=delta_amp  SampleTime=0
  S1b : Step  Time=steer_t1  After=delta_amp  SampleTime=0
  Sat_delta : Saturate  UpperLimit=delta_max  LowerLimit=-delta_max
  Sat_ramp : Saturate  UpperLimit=1  LowerLimit=0
  Sel_modo : MultiPortSwitch  Inputs=5  SaturateOnIntegerOverflow=off  InputSameDT=off
  Sin : Trigonometry
  Sum_tau : Sum  Inputs=+-
  tag scope: delta=global
  wires:
  Clock/1 -> Sum_tau/1
  C_t0/1 -> Sum_tau/2
  S1a/1 -> M1/1
  S1b/1 -> M1/2
  Sum_tau/1 -> G_w/1, G_ramp/1
  G_w/1 -> Sin/1
  Sin/1 -> G_amp/1
  G_amp/1 -> P2/1
  Gate2/1 -> P2/2
  G_ramp/1 -> Sat_ramp/1
  Sat_ramp/1 -> P3/1
  C_R/1 -> P3/2
  C_mode/1 -> Sel_modo/1
  M1/1 -> Sel_modo/2
  P2/1 -> Sel_modo/3
  P3/1 -> Sel_modo/4
  FromWS/1 -> Sel_modo/5
  Sel_modo/1 -> RateLim/1
  RateLim/1 -> Sat_delta/1
  Sat_delta/1 -> [delta]
  [delta_pp] -> Sel_modo/6

== system pwtsimplificado/Monitor DC ==
  Int_E : Integrator
  Potencia DC : MATLAB Function  TreatAsAtomicUnit=on
  T1 : Terminator
  T2 : Terminator
  T3 : Terminator
  wires:
  [Vd] -> Potencia DC/1(Vd)
  [Vq] -> Potencia DC/2(Vq)
  [Idm] -> Potencia DC/3(Idm)
  [Iqm] -> Potencia DC/4(Iqm)
  Potencia DC/1(P_dc) -> T1/1
  Potencia DC/2(I_dc) -> T2/1
  Potencia DC/3(P_recup) -> Int_E/1
  Int_E/1 -> T3/1

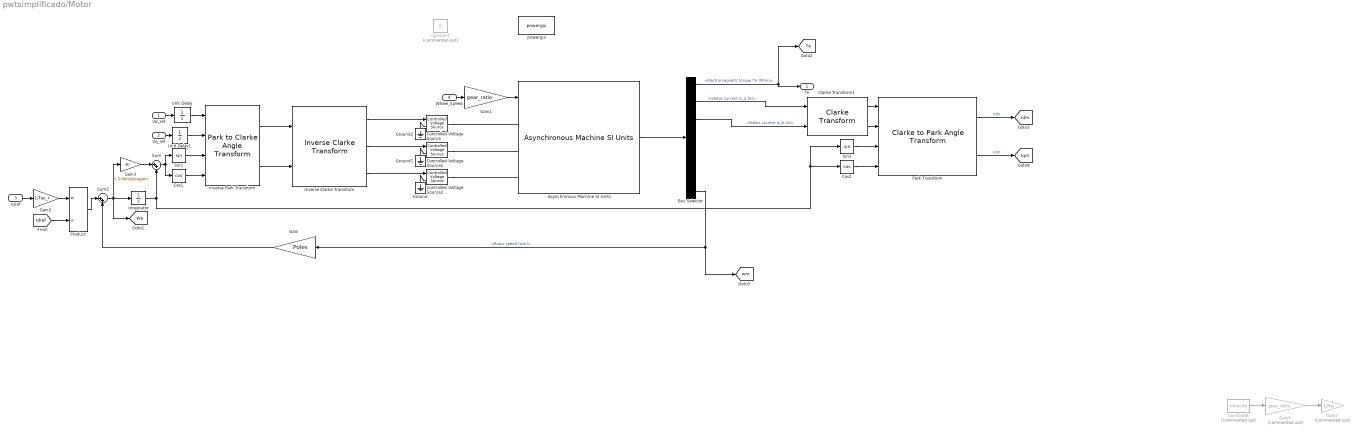
== system pwtsimplificado/Motor ==
  Vd_ref : Inport
  Vq_ref : Inport  Port=2
  Iqref : Inport  Port=3
  Wheel_Speed : Inport  Port=4
  Asynchronous Machine SI Units : spsAsynchronousMachineSIUnitsLib/Asynchronous Machine SI Units  RotorType=Squirrel-cage  PresetModel=No  MechanicalLoad=Speed w  ShowDetailedParameters=on  ReferenceFrame=Stationary  Units=SI  MeasurementBus=off  NominalParameters=[20143, 102, 100]  VoltageRatio=1  Stator=[Rs Lls]  Rotor=[Rr Llr]  Cage1=[0.4155 0.002066]  Cage2=[0.4168 0.0003495]  Lm=Lm  Mechanical=[Im 0.00001 Poles]  PolePairs=2  InitialConditions=[0 0 0 0 0 0 0 0]  SimulateSaturation=off  Saturation=[14.03593122, 27.81365428, 53.79336849, 72.68890987, 97.98006896, 148.6815601, 215.7428561, 302.9841135, 428.7778367 ; 230, 322, 414, 460, 506, 552, 598, 644, 690]  LoadFlowParameters=1492000  TsPowergui=0  TsBlock=Amostragem  IterativeModel=Trapezoidal non iterative  IterativeDiscreteModel=Trapezoidal non iterative  Pmec=Pnom
  Bus Selector : BusSelector  OutputSignals=Mechanical.Electromagnetic torque Te (N*m),Stator measurements.Stator current is_a (A),Stator measurements.Stator current is_b (A),Mechanical.Rotor angle thetam (rad),Rotor measurements.Rotor flux phir_q (V s),Rotor measurements.Rotor flux phir_d (V s),Mechanical.Rotor speed (wm)
  Clarke Transform1 : mcbeeMathTransformLib/Clarke Transform  VariantControl=Variant2  PowerInvariant=off  UseWithEmbedded=on  PhaseInput=Two inputs
      settings: LibrarySourceBlock=mcbcontrolslib/Clarke Transform
  Constant : Constant  Commented=on  Value=0
  Constant8 : Constant  Commented=on  Value=Velocity
  Controlled Voltage Source : spsControlledVoltageSourceLib/Controlled Voltage Source  Initialize=on  Source_Type=AC  Amplitude=0  Phase=0  Frequency=0  Measurements=None
  Controlled Voltage Source1 : spsControlledVoltageSourceLib/Controlled Voltage Source  Initialize=on  Source_Type=AC  Amplitude=0  Phase=0  Frequency=0  Measurements=None
  Controlled Voltage Source2 : spsControlledVoltageSourceLib/Controlled Voltage Source  Initialize=on  Source_Type=AC  Amplitude=0  Phase=0  Frequency=0  Measurements=None
  Cos1 : Trigonometry  Operator=cos
  Cos2 : Trigonometry  Operator=cos
  Gain : Gain  Gain=Poles
  Gain1 : Gain  Gain=gear_ratio
  Gain2 : Gain  Gain=1/Tau_r
  Gain3 : Gain  Gain=1.5*Amostragem
  Gain6 : Gain  Commented=on  Gain=gear_ratio
  Gain7 : Gain  Commented=on  Gain=1/Rw
  Ground : spsGroundLib/Ground  LConnTagsString=a
  Ground1 : spsGroundLib/Ground  LConnTagsString=a
  Ground2 : spsGroundLib/Ground  LConnTagsString=a
  Integrator : Integrator  WrapState=on  WrappedStateUpperValue=2*pi  WrappedStateLowerValue=0
  Inverse Clarke Transform : mcbeeMathTransformLib/Inverse Clarke Transform  PowerInvariant=off  UseWithEmbedded=on  PhaseInput=Two inputs
      settings: LibrarySourceBlock=mcbcontrolslib/Inverse Clarke Transform
  Inverse Park Transform : mcbeeMathTransformLib/Park to Clarke Angle Transform  AxisAlignment=D-axis  UseWithEmbedded=on  PhaseInput=Two inputs  ThetaInput=Sine and Cosine electrical position  AngleInput=Per-unit  N_points=1024
      settings: LibrarySourceBlock=mcbcontrolslib/Inverse Park Transform
  Park Transform : mcbeeMathTransformLib/Clarke to Park Angle Transform  AxisAlignment=D-axis  UseWithEmbedded=on  PhaseInput=Two inputs  ThetaInput=Sine and Cosine electrical position  AngleInput=Per-unit  N_points=1024
      settings: LibrarySourceBlock=mcbcontrolslib/Park Transform
  Product : Product  Inputs=*/
  Sin1 : Trigonometry
  Sin2 : Trigonometry
  Sum : Sum  Inputs=|++
  Sum2 : Sum  Inputs=|++
  Unit Delay : UnitDelay  SampleTime=Amostragem  HasFrameUpgradeWarning=on
  Unit Delay1 : UnitDelay  SampleTime=Amostragem  HasFrameUpgradeWarning=on
  powergui : spspowerguiLib/powergui  Priority=1  SimulationMode=Discrete  SampleTime=Amostragem  frequency=60  Iterations=50  frequencyindice=0  Pbase=100e6  ErrMax=1e-4  UnitsV=kV  UnitsW=MW  buscounter=0  FunctionMessages=off  echomessages=off  EnableUseOfTLC=off  CurrentSourceSwitches=off  DisableSnubberDevices=off  DisableRonSwitches=off  DisableVfSwitches=off  DisplayEquations=off  AutomaticDiscreteSolvers=off  SolverType=Tustin/Backward Euler (TBE)  Interpol=off  ExternalGateDelay=off  methode=off  Ts=100  x0status=blocks  SPID=on  SwTol=0  HookPort=off  NonlinearTolerance=1e-4  nMaxIteration=100  ContinueOnMaxIteration=off  RestoreLinks=warning  ResistiveCurrentMeasurement=off  Frange=[0:2:500]  Ylog=off  Xlog=on  ShowGrid=off  save=off  variable=ZData  structure=0  ZoomFFT=off  StartTime=0.0  cycles=1  DisplayStyle=1  fundamental=60  FreqAxis=off  MaxFrequency=1000  frequencyindicesteady=1  RmsSteady=1  display=off
  Te : Outport
  tag scope: Idm=global, Iqm=global, Te=global, We=global, wm=global
  wires:
  Inverse Park Transform/1 -> Inverse Clarke Transform/1
  Inverse Park Transform/2 -> Inverse Clarke Transform/2
  Asynchronous Machine SI Units/1 -> Bus Selector/1
  Bus Selector/1 -> Te/1, [Te]  "<Electromagnetic torque Te (N*m)>"
  Clarke Transform1/2 -> Park Transform/2
  Clarke Transform1/1 -> Park Transform/1
  Bus Selector/2 -> Clarke Transform1/1  "<Stator current is_a (A)>"
  Bus Selector/3 -> Clarke Transform1/2  "<Stator current is_b (A)>"
  Integrator/1 -> Sin2/1, Cos2/1, Sum/2
  Park Transform/1 -> [Idm]  "Idm"
  Park Transform/2 -> [Iqm]  "Iqm"
  Inverse Clarke Transform/2 -> Controlled Voltage Source1/1
  Inverse Clarke Transform/3 -> Controlled Voltage Source2/1
  Iqref/1 -> Gain2/1
  Gain2/1 -> Product/1
  Product/1 -> Sum2/1
  Gain6/1 -> Gain7/1
  Constant8/1 -> Gain6/1
  Sum2/1 -> Integrator/1, [We], Gain3/1
  Inverse Clarke Transform/1 -> Controlled Voltage Source/1
  Bus Selector/7 -> [wm], Gain/1  "<Rotor speed (wm)>"
  Unit Delay/1 -> Inverse Park Transform/1
  Unit Delay1/1 -> Inverse Park Transform/2
  [Idref] -> Product/2
  Vq_ref/1 -> Unit Delay1/1
  Vd_ref/1 -> Unit Delay/1
  Gain/1 -> Sum2/2
  Wheel_Speed/1 -> Gain1/1
  Gain1/1 -> Asynchronous Machine SI Units/1
  Cos1/1 -> Inverse Park Transform/4
  Sin1/1 -> Inverse Park Transform/3
  Gain3/1 -> Sum/1
  Sum/1 -> Cos1/1, Sin1/1
  Sin2/1 -> Park Transform/3
  Cos2/1 -> Park Transform/4
  connections:
  Controlled Voltage Source/RConn1 -- Asynchronous Machine SI Units/LConn1
  Controlled Voltage Source1/RConn1 -- Asynchronous Machine SI Units/LConn2
  Controlled Voltage Source2/RConn1 -- Asynchronous Machine SI Units/LConn3
  Ground/LConn1 -- Controlled Voltage Source2/LConn1
  Ground1/LConn1 -- Controlled Voltage Source1/LConn1
  Ground2/LConn1 -- Controlled Voltage Source/LConn1

== system pwtsimplificado/Piloto ==
  PurePursuit : MATLAB Function  TreatAsAtomicUnit=on
  T1 : Terminator
  tag scope: delta_pp=global, frn_pp=global, ped_pp=global
  wires:
  [X_pos] -> PurePursuit/1(X)
  [Y_pos] -> PurePursuit/2(Y)
  PurePursuit/1(delta) -> [delta_pp]
  [psi] -> PurePursuit/3(psi)
  [Velocity] -> PurePursuit/4(Vx)
  PurePursuit/2(ped) -> [ped_pp]
  PurePursuit/3(frn) -> [frn_pp]
  PurePursuit/4(v_alvo) -> T1/1

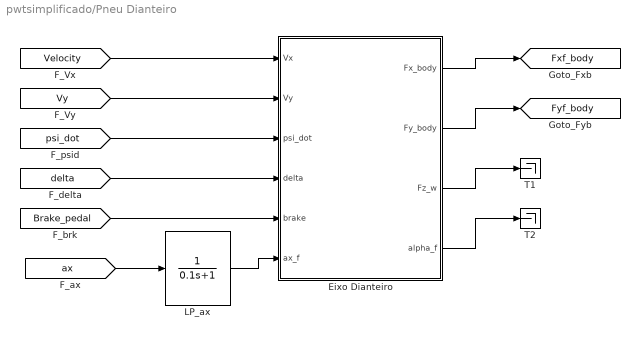
== system pwtsimplificado/Pneu Dianteiro ==
  Eixo Dianteiro : MATLAB Function  TreatAsAtomicUnit=on
  LP_ax : TransferFcn  Denominator=[0.1 1]
  T1 : Terminator
  T2 : Terminator
  tag scope: Fxf_body=global, Fyf_body=global
  wires:
  [Velocity] -> Eixo Dianteiro/1(Vx)
  [Vy] -> Eixo Dianteiro/2(Vy)
  [psi_dot] -> Eixo Dianteiro/3(psi_dot)
  [delta] -> Eixo Dianteiro/4(delta)
  [Brake_pedal] -> Eixo Dianteiro/5(brake)
  [ax] -> LP_ax/1
  LP_ax/1 -> Eixo Dianteiro/6(ax_f)
  Eixo Dianteiro/1(Fx_body) -> [Fxf_body]
  Eixo Dianteiro/2(Fy_body) -> [Fyf_body]
  Eixo Dianteiro/3(Fz_w) -> T1/1
  Eixo Dianteiro/4(alpha_f) -> T2/1

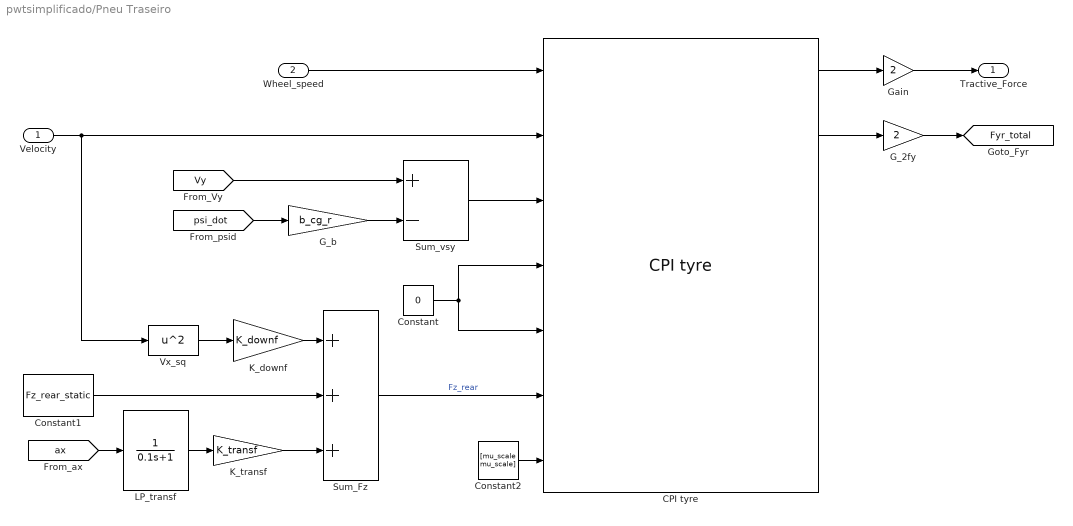
== system pwtsimplificado/Pneu Traseiro ==
  Velocity : Inport
  Wheel_speed : Inport  Port=2
  CPI tyre : mfeval_LIB/CPI tyre  Description=Magic Formula 6.1.2 tyre model including relaxation length and transient calculations  userParameterSource=tirParams  userSide=1 left  userDynamics=1 steady state  userUseMode=1 combined  enablePressure=off  userPressure=2.3
      settings: SourceProductName=MFeval Library
  Constant : Constant  Value=0
  Constant1 : Constant  Value=Fz_rear_static
  Constant2 : Constant  Value=[mu_scale mu_scale]
  G_2fy : Gain  Gain=2
  G_b : Gain  Gain=b_cg_r
  Gain : Gain  Gain=2
  K_downf : Gain  Gain=K_downf
  K_transf : Gain  Gain=K_transf
  LP_transf : TransferFcn  Denominator=[0.1 1]
  Sum_Fz : Sum  Inputs=+++
  Sum_vsy : Sum  Inputs=+-
  Vx_sq : Math  Operator=square
  Tractive_Force : Outport
  tag scope: Fyr_total=global
  wires:
  Constant/1 -> CPI tyre/4, CPI tyre/5
  Constant2/1 -> CPI tyre/7
  CPI tyre/1 -> Gain/1
  Velocity/1 -> Vx_sq/1, CPI tyre/2
  Wheel_speed/1 -> CPI tyre/1
  Gain/1 -> Tractive_Force/1
  Constant1/1 -> Sum_Fz/2
  K_transf/1 -> Sum_Fz/3
  Vx_sq/1 -> K_downf/1
  K_downf/1 -> Sum_Fz/1
  Sum_Fz/1 -> CPI tyre/6  "Fz_rear"
  [ax] -> LP_transf/1
  LP_transf/1 -> K_transf/1
  [Vy] -> Sum_vsy/1
  [psi_dot] -> G_b/1
  G_b/1 -> Sum_vsy/2
  Sum_vsy/1 -> CPI tyre/3
  CPI tyre/2 -> G_2fy/1
  G_2fy/1 -> [Fyr_total]

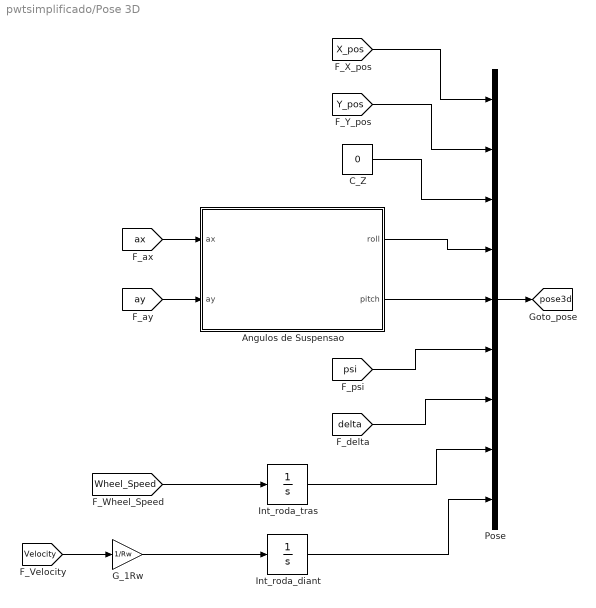
== system pwtsimplificado/Pose 3D ==
  Angulos de Suspensao : MATLAB Function  TreatAsAtomicUnit=on
  C_Z : Constant  Value=0
  G_1Rw : Gain  Gain=1/Rw
  Int_roda_diant : Integrator
  Int_roda_tras : Integrator
  Pose : Mux  Inputs=9
  tag scope: pose3d=global
  wires:
  G_1Rw/1 -> Int_roda_diant/1
  [Velocity] -> G_1Rw/1
  [Wheel_Speed] -> Int_roda_tras/1
  [psi] -> Pose/6
  [ax] -> Angulos de Suspensao/1(ax)
  [X_pos] -> Pose/1
  [delta] -> Pose/7
  [ay] -> Angulos de Suspensao/2(ay)
  [Y_pos] -> Pose/2
  C_Z/1 -> Pose/3
  Angulos de Suspensao/1(roll) -> Pose/4
  Angulos de Suspensao/2(pitch) -> Pose/5
  Int_roda_tras/1 -> Pose/8
  Int_roda_diant/1 -> Pose/9
  Pose/1 -> [pose3d]

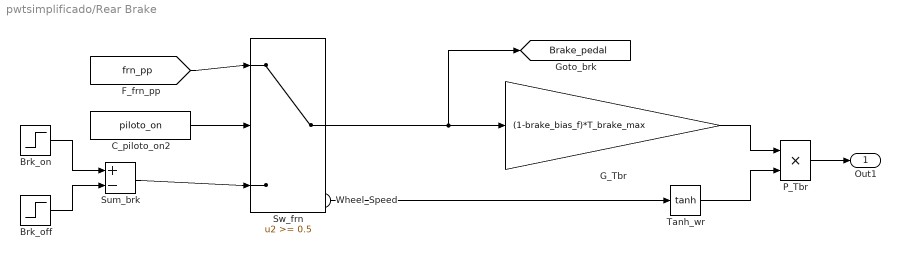
== system pwtsimplificado/Rear Brake ==
  Wheel_Speed : Inport
  Brk_off : Step  Time=11.5  After=0.6  SampleTime=0
  Brk_on : Step  Time=9.5  After=0.6  SampleTime=0
  C_piloto_on2 : Constant  Value=piloto_on
  G_Tbr : Gain  Gain=(1-brake_bias_f)*T_brake_max
  P_Tbr : Product
  Sum_brk : Sum  Inputs=+-
  Sw_frn : Switch  Threshold=0.5
  Tanh_wr : Trigonometry  Operator=tanh
  Out1 : Outport
  tag scope: Brake_pedal=global
  wires:
  Brk_off/1 -> Sum_brk/2
  Brk_on/1 -> Sum_brk/1
  G_Tbr/1 -> P_Tbr/1
  Wheel_Speed/1 -> Tanh_wr/1
  Sw_frn/1 -> G_Tbr/1, [Brake_pedal]
  Tanh_wr/1 -> P_Tbr/2
  P_Tbr/1 -> Out1/1
  [frn_pp] -> Sw_frn/1
  C_piloto_on2/1 -> Sw_frn/2
  Sum_brk/1 -> Sw_frn/3

== system pwtsimplificado/Regen ==
  T_accel : Inport
  Logica Regen : MATLAB Function  TreatAsAtomicUnit=on
  Rampa Regen : RateLimiter  RisingSlewLimit=regen_rate  FallingSlewLimit=-regen_rate  SampleTimeMode=inherited
  Sw_regen : Switch  Criteria=u2 > Threshold  Threshold=0.5  SaturateOnIntegerOverflow=off  InputSameDT=off
  Torque_ref : Outport
  wires:
  [Pedal_accel] -> Logica Regen/1(pedal)
  [Velocity] -> Logica Regen/2(Vx)
  [wm] -> Logica Regen/3(wm)
  Logica Regen/1(T_regen) -> Rampa Regen/1
  Rampa Regen/1 -> Sw_regen/1
  Logica Regen/2(acel_solto) -> Sw_regen/2
  T_accel/1 -> Sw_regen/3
  Sw_regen/1 -> Torque_ref/1

== system pwtsimplificado/Segurança do Pedal ==
  T_pedal : Inport
  C_um : Constant
  G_bcut : Gain  Gain=1/brake_cut
  P_gate : Product
  Sat_gate : Saturate  UpperLimit=1  LowerLimit=0
  Sum_gate : Sum  Inputs=+-
  T_accel : Outport
  wires:
  Sat_gate/1 -> P_gate/2
  [Brake_pedal] -> G_bcut/1
  Sum_gate/1 -> Sat_gate/1
  C_um/1 -> Sum_gate/1
  G_bcut/1 -> Sum_gate/2
  T_pedal/1 -> P_gate/1
  P_gate/1 -> T_accel/1

== system pwtsimplificado/Signal Builder1 ==
  Demux : Demux  Tag=STV Demux  Outputs=1
      settings: DisplayOption=none
  FromWs : FromWorkspace  Tag=STV FromWs  VariableName=tuvar
      SigBuilderData=|
      | common.afterFinalStr = 'Extrapolate'
      | common.sampleTime = 0
      | dataSet.timeRange = [0 12]
      | dataSet.name = 'Group 1'
      | sbobj.Groups.Name = 'Group 1'
      | sbobj.Groups.Signals.Name = 'Signal 1'
      | sbobj.Groups.Signals.XData = [0 0.1 7 7.05 12]
      | sbobj.Groups.Signals.YData = [0.5 100 100 0 0]
      | sbobj.Groups.TimeRange = [0 12]
  Signal 1 : Outport  Tag=STV Outport
  wires:
  Demux/1 -> Signal 1/1
  FromWs/1 -> Demux/1

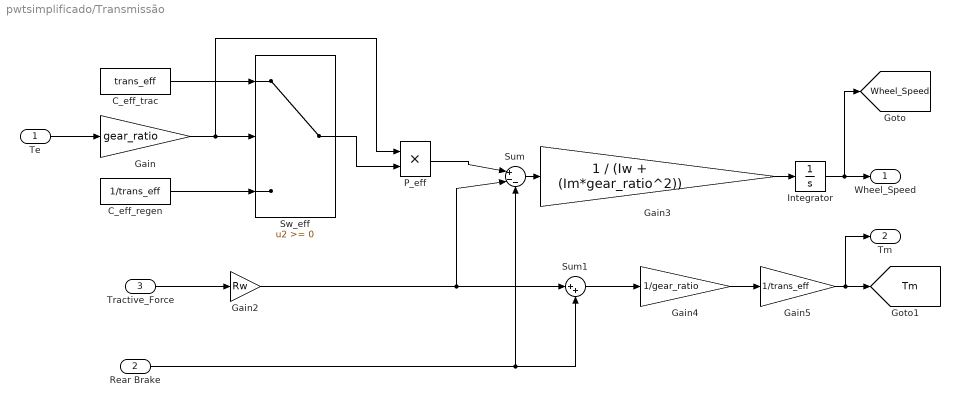
== system pwtsimplificado/Transmissão ==
  Te : Inport
  Rear Brake : Inport  Port=2
  Tractive_Force : Inport  Port=3
  C_eff_regen : Constant  Value=1/trans_eff
  C_eff_trac : Constant  Value=trans_eff
  Gain : Gain  Gain=gear_ratio
  Gain2 : Gain  Gain=Rw
  Gain3 : Gain  Gain=1 / (Iw + (Im*gear_ratio^2))
  Gain4 : Gain  Gain=1/gear_ratio
  Gain5 : Gain  Gain=1/trans_eff
  Integrator : Integrator
  P_eff : Product
  Sum : Sum  Inputs=|+--
  Sum1 : Sum  Inputs=|++
  Sw_eff : Switch  SaturateOnIntegerOverflow=off  InputSameDT=off
  Wheel_Speed : Outport
  Tm : Outport  Port=2
  tag scope: Tm=global, Wheel_Speed=global
  wires:
  Tractive_Force/1 -> Gain2/1
  Gain2/1 -> Sum/2, Sum1/1
  Gain3/1 -> Integrator/1
  Sum/1 -> Gain3/1
  Rear Brake/1 -> Sum/3, Sum1/2
  Integrator/1 -> [Wheel_Speed], Wheel_Speed/1
  Gain4/1 -> Gain5/1
  Sum1/1 -> Gain4/1
  Gain5/1 -> Tm/1, [Tm]
  Te/1 -> Gain/1
  Gain/1 -> Sw_eff/2, P_eff/1
  C_eff_trac/1 -> Sw_eff/1
  C_eff_regen/1 -> Sw_eff/3
  Sw_eff/1 -> P_eff/2
  P_eff/1 -> Sum/1

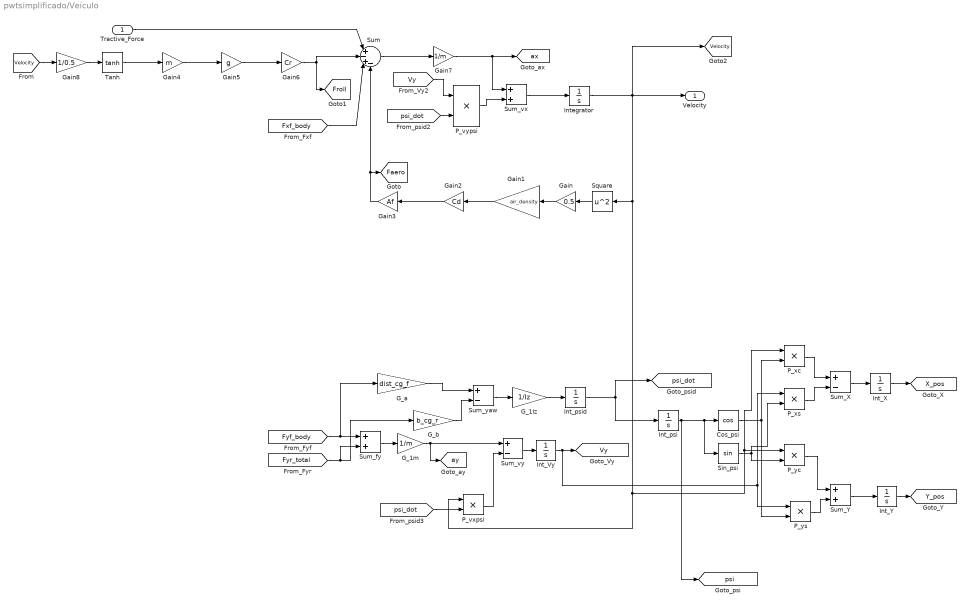
== system pwtsimplificado/Veículo ==
  Tractive_Force : Inport
  Cos_psi : Trigonometry  Operator=cos
  G_1Iz : Gain  Gain=1/Iz
  G_1m : Gain  Gain=1/m
  G_a : Gain  Gain=dist_cg_f
  G_b : Gain  Gain=b_cg_r
  Gain : Gain  Gain=0.5
  Gain1 : Gain  Gain=air_density
  Gain2 : Gain  Gain=Cd
  Gain3 : Gain  Gain=Af
  Gain4 : Gain  Gain=m
  Gain5 : Gain  Gain=g
  Gain6 : Gain  Gain=Cr
  Gain7 : Gain  Gain=1/m
  Gain8 : Gain  Gain=1/0.5
  Int_Vy : Integrator
  Int_X : Integrator
  Int_Y : Integrator
  Int_psi : Integrator
  Int_psid : Integrator
  Integrator : Integrator
  P_vxpsi : Product
  P_vypsi : Product
  P_xc : Product
  P_xs : Product
  P_yc : Product
  P_ys : Product
  Sin_psi : Trigonometry
  Square : Math  Operator=square
  Sum : Sum  Inputs=|+-+-
  Sum_X : Sum  Inputs=+-
  Sum_Y : Sum
  Sum_fy : Sum
  Sum_vx : Sum
  Sum_vy : Sum  Inputs=+-
  Sum_yaw : Sum  Inputs=+-
  Tanh : Trigonometry  Operator=tanh
  Velocity : Outport
  tag scope: Faero=global, Froll=global, Velocity=global, Vy=global, X_pos=global, Y_pos=global, ax=global, ay=global, psi=global, psi_dot=global
  wires:
  Integrator/1 -> Velocity/1, P_xc/1, P_yc/1, P_vxpsi/1, Square/1, [Velocity]
  Gain5/1 -> Gain6/1
  Gain4/1 -> Gain5/1
  Tanh/1 -> Gain4/1
  Gain2/1 -> Gain3/1
  Gain1/1 -> Gain2/1
  Gain/1 -> Gain1/1
  Square/1 -> Gain/1
  Tractive_Force/1 -> Sum/1
  Gain6/1 -> [Froll], Sum/2
  Gain3/1 -> Sum/4, [Faero]
  Sum/1 -> Gain7/1
  Gain7/1 -> Sum_vx/1, [ax]
  [Velocity] -> Gain8/1
  Gain8/1 -> Tanh/1
  [Fxf_body] -> Sum/3
  P_vypsi/1 -> Sum_vx/2
  Sum_vx/1 -> Integrator/1
  [Fyf_body] -> G_a/1, Sum_fy/1
  [Fyr_total] -> Sum_fy/2, G_b/1
  Sum_fy/1 -> G_1m/1
  G_1m/1 -> Sum_vy/1, [ay]
  P_vxpsi/1 -> Sum_vy/2
  Sum_vy/1 -> Int_Vy/1
  Int_Vy/1 -> P_xs/1, P_ys/1, [Vy]
  G_a/1 -> Sum_yaw/1
  G_b/1 -> Sum_yaw/2
  Sum_yaw/1 -> G_1Iz/1
  G_1Iz/1 -> Int_psid/1
  Int_psid/1 -> Int_psi/1, [psi_dot]
  [Vy] -> P_vypsi/1
  [psi_dot] -> P_vypsi/2
  [psi_dot] -> P_vxpsi/2
  Int_psi/1 -> Sin_psi/1, Cos_psi/1, [psi]
  Cos_psi/1 -> P_xc/2, P_ys/2
  Sin_psi/1 -> P_xs/2, P_yc/2
  P_xc/1 -> Sum_X/1
  P_xs/1 -> Sum_X/2
  P_yc/1 -> Sum_Y/1
  P_ys/1 -> Sum_Y/2
  Sum_X/1 -> Int_X/1
  Sum_Y/1 -> Int_Y/1
  Int_X/1 -> [X_pos]
  Int_Y/1 -> [Y_pos]

== system pwtsimplificado/Controladores/Cálculo Saturação Eixo Q ==
  Id_ref : Inport
  Constant : Constant  Value=I_max^2
  Constant1 : Constant  Value=0
  MinMax : MinMax  Function=max  Inputs=2
  Sqrt : Sqrt
  Square : Math  Operator=square
  Sum2 : Sum  Inputs=|-+
  tag scope: Iq_sat=global
  wires:
  Constant/1 -> Sum2/2
  Square/1 -> Sum2/1
  Id_ref/1 -> Square/1
  Sum2/1 -> MinMax/1
  Constant1/1 -> MinMax/2
  MinMax/1 -> Sqrt/1
  Sqrt/1 -> [Iq_sat]

== system pwtsimplificado/Controladores/Feed Forward eixo D ==
  FF_Vd : Scope
      settings: ActiveDisplayYMinimum=-29.823375414585424  ActiveDisplayYMaximum=39.827740751572378  DataLoggingMaxPoints=500000  DataLoggingVariableName=ScopeData9
  Gain3 : Gain  Gain=sigma
  Gain4 : Gain  Gain=Ls
  Product : Product
  We*Iqm*sigma*Ls : Outport
  tag scope: FF=global
  wires:
  Gain3/1 -> Gain4/1
  [Iqm] -> Product/2
  Product/1 -> Gain3/1
  [We] -> Product/1
  Gain4/1 -> [FF], FF_Vd/1, We*Iqm*sigma*Ls/1

== system pwtsimplificado/Controladores/Feed Forward eixo Q ==
  note: Back EMF
  Back-Emf : Scope
      settings: ActiveDisplayYMinimum=-1218.68613  ActiveDisplayYMaximum=190.7559  DataLoggingMaxPoints=500000
  Gain : Gain  Gain=sigma
  Gain1 : Gain  Gain=Ls
  Gain12 : Gain  Gain=(Lm^2)/Lr
  Product1 : Product
  Sum4 : Sum  Inputs=|++
  Back-emf : Outport
  tag scope: Back_Emf=global
  wires:
  Gain/1 -> Gain1/1
  Gain12/1 -> Sum4/2
  [We] -> Product1/2
  Product1/1 -> Gain12/1, Gain/1
  Gain1/1 -> Sum4/1
  [Idm] -> Product1/1
  Sum4/1 -> Back-emf/1, [Back_Emf], Back-Emf/1

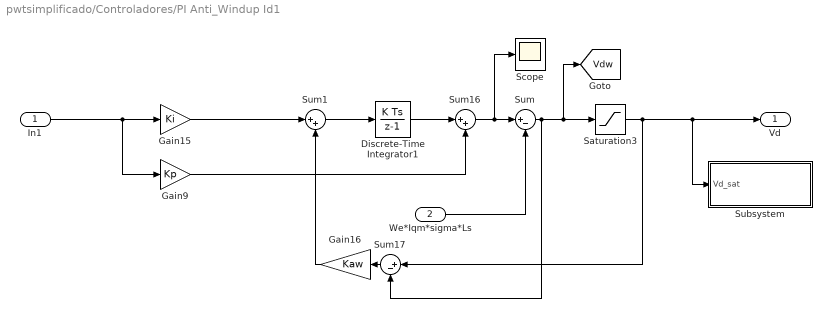
== system pwtsimplificado/Controladores/PI Anti_Windup Id1 ==
  In1 : Inport
  We*Iqm*sigma*Ls : Inport  Port=2
  Discrete-Time Integrator1 : DiscreteIntegrator  SampleTime=Amostragem  ICPrevOutput=DiscIntNeverNeededParam  ICPrevScaledInput=DiscIntNeverNeededParam
  Gain15 : Gain  Gain=Ki
  Gain16 : Gain  Gain=Kaw
  Gain9 : Gain  Gain=Kp
  Saturation3 : Saturate  UpperLimit=(Bv*Modulation_Target)/sqrt(3)  LowerLimit=-(Bv*Modulation_Target)/sqrt(3)
  Scope : Scope
      settings: ActiveDisplayYMinimum=1.3114775524509457  ActiveDisplayYMaximum=7.0252862645949152  DataLoggingVariableName=ScopeData15
  Subsystem : Subsystem
  Sum : Sum  Inputs=|+-
  Sum1 : Sum  Inputs=|++
  Sum16 : Sum  Inputs=|++
  Sum17 : Sum  Inputs=|+-
  Vd : Outport
  tag scope: Vdw=global
  wires:
  Sum1/1 -> Discrete-Time Integrator1/1
  Sum17/1 -> Gain16/1
  Gain9/1 -> Sum16/2
  Saturation3/1 -> Subsystem/1(Vd_sat), Vd/1, Sum17/1
  In1/1 -> Gain15/1, Gain9/1
  Sum16/1 -> Scope/1, Sum/1
  Sum/1 -> Sum17/2, [Vdw], Saturation3/1
  We*Iqm*sigma*Ls/1 -> Sum/2
  Gain15/1 -> Sum1/1
  Gain16/1 -> Sum1/2
  Discrete-Time Integrator1/1 -> Sum16/1

== system pwtsimplificado/Controladores/PI Anti_Windup Id2 ==
  In1 : Inport
  Discrete-Time Integrator1 : DiscreteIntegrator  SampleTime=Amostragem  ICPrevOutput=DiscIntNeverNeededParam  ICPrevScaledInput=DiscIntNeverNeededParam
  Gain15 : Gain  Gain=Ki_fw
  Gain16 : Gain  Gain=Kaw_fw
  Gain9 : Gain  Gain=Kp_fw
  Saturation3 : Saturate  UpperLimit=dImag_max  LowerLimit=dImag_min
  Scope : Scope
      settings: ActiveDisplayYMinimum=1.3114775524509457  ActiveDisplayYMaximum=7.0252862645949152  DataLoggingVariableName=ScopeData15
  Sum1 : Sum  Inputs=|++
  Sum16 : Sum  Inputs=|++
  Sum17 : Sum  Inputs=|+-
  Fw : Outport
  wires:
  Sum1/1 -> Discrete-Time Integrator1/1
  Sum17/1 -> Gain16/1
  Gain9/1 -> Sum16/2
  Saturation3/1 -> Fw/1, Sum17/1
  In1/1 -> Gain15/1, Gain9/1
  Sum16/1 -> Sum17/2, Saturation3/1, Scope/1
  Gain15/1 -> Sum1/1
  Gain16/1 -> Sum1/2
  Discrete-Time Integrator1/1 -> Sum16/1

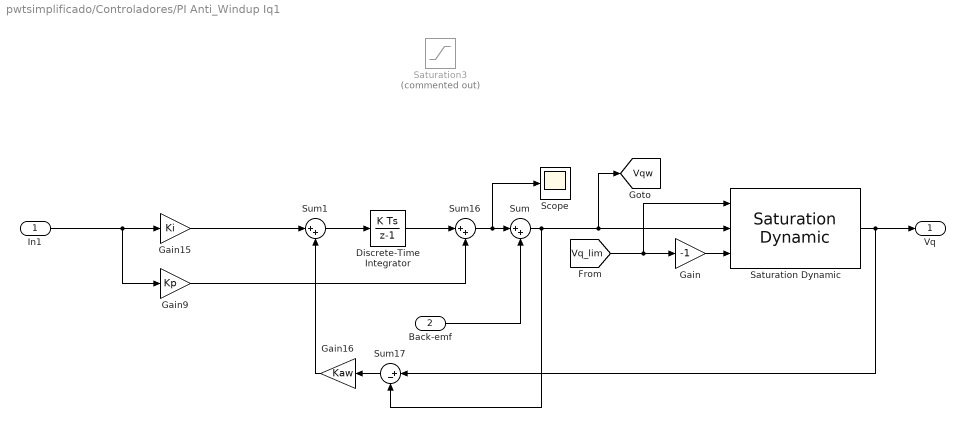
== system pwtsimplificado/Controladores/PI Anti_Windup Iq1 ==
  In1 : Inport
  Back-emf : Inport  Port=2
  Discrete-Time Integrator : DiscreteIntegrator  SampleTime=Amostragem  ICPrevOutput=DiscIntNeverNeededParam  ICPrevScaledInput=DiscIntNeverNeededParam
  Gain : Gain  Gain=-1
  Gain15 : Gain  Gain=Ki
  Gain16 : Gain  Gain=Kaw
  Gain9 : Gain  Gain=Kp
  Saturation Dynamic : simulink/Discontinuities/Saturation Dynamic  OutMin=[]  OutMax=[]  OutDataTypeStr=Inherit: Same as second input  OutDataType=fixdt(1, 16)  OutScaling=2^-10  DoSatur=off
  Saturation3 : Saturate  Commented=on  UpperLimit=Vq_lim  LowerLimit=-Vq_lim
  Scope : Scope
      settings: ActiveDisplayYMinimum=-1.055327868852459  ActiveDisplayYMaximum=3.944672131147541  DataLoggingVariableName=ScopeData14
  Sum : Sum  Inputs=|++
  Sum1 : Sum  Inputs=|++
  Sum16 : Sum  Inputs=|++
  Sum17 : Sum  Inputs=|+-
  Vq : Outport
  tag scope: Vqw=global
  wires:
  Sum1/1 -> Discrete-Time Integrator/1
  Sum17/1 -> Gain16/1
  Gain9/1 -> Sum16/2
  Saturation Dynamic/1 -> Vq/1, Sum17/1
  In1/1 -> Gain15/1, Gain9/1
  Sum16/1 -> Scope/1, Sum/1
  Sum/1 -> [Vqw], Saturation Dynamic/2, Sum17/2
  Back-emf/1 -> Sum/2
  Gain15/1 -> Sum1/1
  Gain16/1 -> Sum1/2
  Discrete-Time Integrator/1 -> Sum16/1
  Gain/1 -> Saturation Dynamic/3
  [Vq_lim] -> Saturation Dynamic/1, Gain/1

== system pwtsimplificado/Controladores/PI Anti_Windup Id1/Subsystem ==
  Vd_sat : Inport
  Constant : Constant  Value=Vmax^2
  Constant1 : Constant  Value=0
  MinMax : MinMax  Function=max  Inputs=2
  Sqrt : Sqrt
  Square : Math  Operator=square
  Sum2 : Sum  Inputs=|-+
  tag scope: Vq_lim=global
  wires:
  Constant/1 -> Sum2/2
  Square/1 -> Sum2/1
  Vd_sat/1 -> Square/1
  Sum2/1 -> MinMax/1
  Constant1/1 -> MinMax/2
  MinMax/1 -> Sqrt/1
  Sqrt/1 -> [Vq_lim]

== matlab function pwtsimplificado/Pose 3D/Angulos de Suspensao ==
  data: ax input; roll output; ay input; pitch output; roll_grad parameter double size=1; pitch_grad parameter double size=1
function [roll, pitch] = fcn(ax, ay, roll_grad, pitch_grad)
%#codegen
% Roll e pitch SINTETIZADOS pelos gradientes quase-estaticos. O modelo tem
% 3 GDL no plano - nao ha dinamica de rolagem nem de arfagem aqui. Serve para
% a visualizacao 3D parecer certa; NAO tire conclusoes de dinamica destes angulos.
g = 9.81;
roll  = -deg2rad(roll_grad)  * (ay/g);   % curva a esquerda (ay>0) -> carro inclina p/ fora
pitch = -deg2rad(pitch_grad) * (ax/g);   % acelerando -> nariz sobe; freando -> mergulha

== matlab function pwtsimplificado/Piloto/PurePursuit ==
  settings: updateMethod=DISCRETE  sampleTime=pp_Ts
  data: X input; delta output; Y input; psi input; Vx input; ped output; frn output; v_alvo output; trk_x parameter; trk_y parameter; trk_k parameter; trk_passo parameter; pp_Ld_min parameter; pp_Ld_k parameter; pp_v_max parameter; pp_ay_max parameter; pp_kp_v parameter; pp_prev parameter; L_wb parameter; pp_ped_max parameter; pp_kp_b parameter; pp_v_banda parameter; pp_frn_max parameter
function [delta, ped, frn, v_alvo] = fcn(X, Y, psi, Vx, trk_x, trk_y, trk_k, trk_passo, pp_Ld_min, pp_Ld_k, pp_v_max, pp_ay_max, pp_kp_v, pp_prev, L_wb, pp_ped_max, pp_kp_b, pp_v_banda, pp_frn_max)
%#codegen
% Piloto de pure pursuit. Roda em tempo discreto e guarda o indice do ultimo
% ponto mais proximo, o que permite buscar so numa JANELA a frente em vez de
% varrer a pista inteira a cada passo - com ~530 pontos e passo de 12,5 us a
% busca completa dominaria o custo da simulacao.

persistent i0
if isempty(i0)
    i0 = int32(1);
end
N = int32(numel(trk_x));

% --- 1. ponto mais proximo, procurando so para a frente ---
% So para a frente de proposito: impede o piloto de 'voltar' e travar quando a
% pista passa perto dela mesma.
melhor = inf;
ib = i0;
for j = int32(0):int32(60)
    id = mod(i0 - 1 + j, N) + 1;
    d2 = (trk_x(id) - X)^2 + (trk_y(id) - Y)^2;
    if d2 < melhor
        melhor = d2;
        ib = id;
    end
end
i0 = ib;

% --- 2. ponto de mira ---
% Ld cresce com a velocidade: perto do carro em baixa (precisao), longe em alta
% (estabilidade). Ld fixo da serpente em reta ou corta curva, dependendo do valor.
Ld = pp_Ld_min;
if pp_Ld_k * Vx > Ld
    Ld = pp_Ld_k * Vx;
end
n  = int32(round(Ld / trk_passo));
if n < int32(1)
    n = int32(1);
end
it = mod(ib - 1 + n, N) + 1;

% --- 3. a geometria do pure pursuit ---
% alpha e o angulo entre o eixo do carro e a linha ate o ponto de mira. O arco
% que liga os dois tem raio Ld/(2 sin alpha); Ackermann converte raio em esterco.
al = atan2(trk_y(it) - Y, trk_x(it) - X) - psi;
al = atan2(sin(al), cos(al));
delta = atan2(2 * L_wb * sin(al), Ld);

% --- 4. velocidade alvo pela curvatura que vem pela frente ---
% Olha pp_prev metros adiante e pega a curva mais fechada: v = sqrt(ay_max/k).
% E o mesmo criterio de elipse de atrito, so que na versao mais simples.
kmax = 1e-4;
nf = int32(round(pp_prev / trk_passo));
for j = int32(0):nf
    id = mod(ib - 1 + j, N) + 1;
    ak = abs(trk_k(id));
    if ak > kmax
        kmax = ak;
    end
end
v_alvo = sqrt(pp_ay_max / kmax);
if v_alvo > pp_v_max
    v_alvo = pp_v_max;
end

% --- 5. acelerador e freio ---
% DUAS ESCALAS DIFERENTES, e confundi-las nao gera erro nenhum:
%   acelerador: o 'pedal' do modelo e requisicao de TORQUE (lookup [0:94]),
%               entao a fracao 0..1 e multiplicada por pp_ped_max.
%   freio:      o Brake_pedal ja e FRACAO 0..1, vai direto.
% Os dois nunca sao acionados juntos - e um piloto, nao um teste de banco.
err = v_alvo - Vx;
ped = 0;
frn = 0;
if err >= 0
    frac = pp_kp_v * err;
    if frac > 1
        frac = 1;
    end
    ped = frac * pp_ped_max;
elseif err < -pp_v_banda
    % So pisa no freio quando o regen de lift-off nao da conta. A banda morta
    % evita alternar acelerador/freio a cada passo em torno da velocidade alvo,
    % que e o que faz um piloto ruim (e um controlador sem histerese).
    frn = pp_kp_b * (-err - pp_v_banda);
    if frn > pp_frn_max
        frn = pp_frn_max;
    end
end
end

== matlab function pwtsimplificado/Regen/Logica Regen ==
  data: T_regen output; acel_solto output; pedal input; Vx input; wm input; accel_deadzone parameter double size=1; regen_coast parameter double size=1; T_regen_max parameter double size=1; Bv parameter double size=1; Bi_regen parameter double size=1; motor_eff parameter double size=1; mc_eff parameter double size=1; w_motor_min parameter double size=1; v_regen_off parameter double size=1; v_regen_full parameter double size=1; regen_margin parameter double size=1
function [T_regen, acel_solto] = fcn(pedal, Vx, wm, accel_deadzone, regen_coast, T_regen_max, Bv, Bi_regen, motor_eff, mc_eff, w_motor_min, v_regen_off, v_regen_full, regen_margin)
%#codegen
% REGEN DE LIFT-OFF - estrategia do carro real: atua sempre que o ACELERADOR
% esta solto. O pedal de FREIO nao entra aqui; o atrito soma por fora.

acel_solto = double(pedal <= accel_deadzone);

% 1) torque desejado - o ajuste de "sensacao de freio motor"
T_desej = regen_coast * T_regen_max;

% 2) LIMITE DA BATERIA. A potencia de recarga nao pode passar de Bv*Bi_regen.
%    Fluxo mecanico -> eletrico, entao as eficiencias MULTIPLICAM.
%    Em rotacao alta este limite e que manda; em baixa ele e generoso.
w      = max(abs(wm), w_motor_min);
T_batt = regen_margin*(Bv*Bi_regen)/(w*motor_eff*mc_eff);

% 3) FADE em baixa velocidade: regra FSAE e fisica (perto da parada o motor nao
%    gera, e o regen empurraria o carro para tras).
fade = (Vx - v_regen_off)/(v_regen_full - v_regen_off);
fade = min(max(fade,0),1);

% 4) zerado enquanto o acelerador esta pressionado. E o que faz a RAMPA de fora
%    enxergar um degrau de 0 -> T_regen quando o piloto tira o pe (sem isto a
%    rampa fica "carregada" e nao suaviza nada).
T_regen = -min(T_desej, T_batt)*fade*acel_solto;
